simulink model "finalmodel1"  (R2024b)
(part 2 of 9)

      mask TypeOptions ModuleName: User-defined | A10Green Technology A10J-S72-175 | A10Green Technology A10J-S72-180 | A10Green Technology A10J-S72-185 | A10Green Technology A10J-M60-220 | A10Green Technology A10J-M60-225 | A10Green Technology A10J-M60-230 | A10Green Technology A10J-M60-235 | A10Green Technology A10J-M60-240 | A2Peak Power POWER ON P220-6x10 | Aavid Solar ASMS-165P | Aavid Solar ASMS-180M | Aavid Solar ASMS-185M | Aavid Solar ASMS-220P | Aavid Solar ASMS-225M | Aavid Solar ASMS-230M | Aavid Solar ASMS-235M | Aavid Solar ASMS-270P | Aavid Thermalloy ASMP-175M | Aavid Thermalloy ASMP-180M | Ablytek 5MN6C175-A0 | Ablytek 5MN6C180-A0 | Ablytek 5MN6C185-A0 | Ablytek 6PN6A220-A0 | Ablytek 6PN6A225-A0 | Ablytek 6PN6A230-A0 | Ablytek 6PN6A235-A0 | Ablytek 6PN6A240-A0 | Ablytek 6MN6A270 | Ablytek 6MN6A275 | Ablytek 6MN6A280 | Ablytek 6MN6A285 | Ablytek 6MN6A290 | AccuSolar Power ASP610-B230 | Advance Power API-P210 | Advance Power API-P215 | Advance Power API-P220 | Advance Power API-M225 | Advance Power API-P225 | Advance Power API-M230 | Advance Power API-P230 | Advance Power API-M235 | Advance Power API-P235 | Advance Power API-M240 | Advance Power API-P240 | Advance Power API-M245 | Advance Power API-P245 | Advance Power API-M250 | Advance Power API-P250 | Advance Power API-M255 | Advance Power API-P255 | Advance Power API-M260 | Advance Power API-P260 | Advance Power API-M265 | Advance Power API-P265 | Advance Power API-M270 | Advance Power API-P270 | Advance Power API-M275 | Advance Power API-P275 | Advance Power API-M280 | Advance Power API-P280 | Advance Power API-M285 | Advance Power API-P285 | Advance Power API-M290 | Advance Power API-P290 | Advance Power API-M295 | Advance Power API-P295 | Advance Power API-M300 | Advance Power API-P300 | Advance Power API-M305 | Advance Power API-P305 | Advance Power API-M310 | Advance Power API-P310 | Advance Power API-M315 | Advance Power API-P315 | Advance Power API-P320 | Advance Power API-P325 | Advance Power API-M330 | Advance Power API-P330 | Advance Power API-M335 | Advance Power API-P335 | Advance Power API-M340 | Advance Power API-M345 | Advance Power API-M350 | Advance Power API-M355 | Advance Power API-M360 | Advance Power API-M365 | Advance Power API-M370 | Advance Solar Hydro Wind Power API-150 | Advance Solar Hydro Wind Power API-160 | Advance Solar Hydro Wind Power API-165 | Advance Solar Hydro Wind Power API-170 | Advance Solar Hydro Wind Power API-175 | Advance Solar Hydro Wind Power API-180 | Advance Solar Hydro Wind Power API156P-200 | Advance Solar Hydro Wind Power API156P-210 | Advance Solar Hydro Wind Power API156P-220 | Advance Solar Hydro Wind Power API156P-230 | Advanced Renewable Energy AREi-210W-M6-G | Advanced Renewable Energy AREi-215W-M6-G | Advanced Renewable Energy AREi-220W-M6-G | Advanced Renewable Energy AREi-225W-M6-G | Advanced Renewable Energy AREi-230W-M6-G | Advanced Solar Power (Hangzhou) ASP-S1-80 | Aleo Solar P18y250 | Aleo Solar S18y250 | Aleo Solar P18y255 | Aleo Solar S18y255 | Aleo Solar P18y260 | Aleo Solar S18y260 | Aleo Solar P18Y265 | Aleo Solar S18y265 | Aleo Solar S19Y270 | Aleo Solar S79y270 | Aleo Solar P19Y275 | Aleo Solar S19y275 | Aleo Solar S79y275 | Aleo Solar S19y280 | Aleo Solar S59y280 | Aleo Solar S79y280 | Aleo Solar P19Y285 | Aleo Solar S19y285 | Aleo Solar S59y285 | Aleo Solar S79y285 | Aleo Solar P19Y290 | Aleo Solar S19y290 | Aleo Solar S59y290 | Aleo Solar S79Y290 | Aleo Solar P19Y295 | Aleo Solar S19Y295 | Aleo Solar S59Y295 | Aleo Solar S79Y295 | Aleo Solar P19Y300 | Aleo Solar S19Y300 | Aleo Solar S59Y300 | Aleo Solar S79Y300 | Aleo Solar P19Y305 | Aleo Solar S19Y305 | Aleo Solar S59Y305 | Aleo Solar S79Y305 | Aleo Solar P19Y310 | Aleo Solar S19Y310 | Aleo Solar S59Y310 | alfasolar alfasolar P6L60-220 | alfasolar alfasolar P6L60-225 | alfasolar alfasolar P6L60-230 | alfasolar alfasolar P6L60-235 | alfasolar alfasolar M6L60-240 | alfasolar alfasolar P6L60-240 | alfasolar alfasolar M6L60-245 | alfasolar alfasolar P6L60-245 | alfasolar alfasolar M6L60-250 | alfasolar alfasolar P6L60-250 | alfasolar alfasolar M6L60-255 | alfasolar alfasolar M6L60-260 | alfasolar alfasolar M6L60-265 | Alps Technology ATI-S572-175 | Alps Technology ATI-S572-180 | Alps Technology ATI-S572-185 | Alps Technology ATI-M660-220 | Alps Technology ATI-M660-225 | Alps Technology ATI-M660-230 | Alps Technology ATI-M660-235 | Alps Technology ATI-M660-240 | American Solar Wholesale ASW-175M | American Solar Wholesale ASW-180M | American Solar Wholesale ASW-185M | American Solar Wholesale ASW-215P | American Solar Wholesale ASW-220P | American Solar Wholesale ASW-225M | American Solar Wholesale ASW-225P | American Solar Wholesale ASW-230M | American Solar Wholesale ASW-230P | American Solar Wholesale ASW-235M | American Solar Wholesale ASW-235P | American Solar Wholesale ASW-240M-60 | American Solar Wholesale ASW-240P | American Solar Wholesale ASW-245M | American Solar Wholesale ASW-245P | American Solar Wholesale ASW-250M | American Solar Wholesale ASW-250P | American Solar Wholesale ASW-260M | American Solar Wholesale ASW-260P | American Solar Wholesale ASW-265M | American Solar Wholesale ASW-270M | American Solar Wholesale ASW-270P | American Solar Wholesale ASW-275M | American Solar Wholesale ASW-280M | American Solar Wholesale ASW-280P | American Solar Wholesale ASW-285M | American Solar Wholesale ASW-285P | American Solar Wholesale ASW-290M | American Solar Wholesale ASW-290P | American Solar Wholesale ASW-295M | American Solar Wholesale ASW-295P | American Solar Wholesale ASW-300M | American Solar Wholesale ASW-300P | American Solar Wholesale ASW-305P | American Solar Wholesale ASW-310P | American Solar Wholesale ASW-315P | American Value SM240-5M | American Value SM245-5M | American Value SM250-5M | American Value SM255-5M | American Value SM260-5M | Amerisolar-Worldwide Energy and Manufacturing USA Co._ Ltd AS-5M36-165W | Amerisolar-Worldwide Energy and Manufacturing USA Co._ Ltd AS-5M-170W | Amerisolar-Worldwide Energy and Manufacturing USA Co._ Ltd AS-5M36-170W | Amerisolar-Worldwide Energy and Manufacturing USA Co._ Ltd AS-6M24-170W | Amerisolar-Worldwide Energy and Manufacturing USA Co._ Ltd AS-6P24-170W | Amerisolar-Worldwide Energy and Manufacturing USA Co._ Ltd AS-5M-175W | Amerisolar-Worldwide Energy and Manufacturing USA Co._ Ltd AS-5M36-175W | Amerisolar-Worldwide Energy and Manufacturing USA Co._ Ltd AS-6M24-175W | Amerisolar-Worldwide Energy and Manufacturing USA Co._ Ltd AS-6P24-175W | Amerisolar-Worldwide Energy and Manufacturing USA Co._ Ltd AS-5M-180W | Amerisolar-Worldwide Energy and Manufacturing USA Co._ Ltd AS-5M36-180W | Amerisolar-Worldwide Energy and Manufacturing USA Co._ Ltd AS-6M24-180W | Amerisolar-Worldwide Energy and Manufacturing USA Co._ Ltd AS-6P24-180W | Amerisolar-Worldwide Energy and Manufacturing USA Co._ Ltd AS-5M-185W | Amerisolar-Worldwide Energy and Manufacturing USA Co._ Ltd AS-5M36-185W | Amerisolar-Worldwide Energy and Manufacturing USA Co._ Ltd AS-6M24-185W | Amerisolar-Worldwide Energy and Manufacturing USA Co._ Ltd AS-6P24-185W | Amerisolar-Worldwide Energy and Manufacturing USA Co._ Ltd AS-5M-190W | Amerisolar-Worldwide Energy and Manufacturing USA Co._ Ltd AS-6M24-190W | Amerisolar-Worldwide Energy and Manufacturing USA Co._ Ltd AS-6P24-190W | Amerisolar-Worldwide Energy and Manufacturing USA Co._ Ltd AS-6M27-215W | Amerisolar-Worldwide Energy and Manufacturing USA Co._ Ltd AS-6M27-B-215W | Amerisolar-Worldwide Energy and Manufacturing USA Co._ Ltd AS-6M27-220W | Amerisolar-Worldwide Energy and Manufacturing USA Co._ Ltd AS-6M27-B-220W | Amerisolar-Worldwide Energy and Manufacturing USA Co._ Ltd AS-6M30-220W | Amerisolar-Worldwide Energy and Manufacturing USA Co._ Ltd AS-6P30-220W | Amerisolar-Worldwide Energy and Manufacturing USA Co._ Ltd AS-6M27-225W | Amerisolar-Worldwide Energy and Manufacturing USA Co._ Ltd AS-6M27-B-225W | Amerisolar-Worldwide Energy and Manufacturing USA Co._ Ltd AS-6M30-225W | Amerisolar-Worldwide Energy and Manufacturing USA Co._ Ltd AS-6P30-225W | Amerisolar-Worldwide Energy and Manufacturing USA Co._ Ltd AS-6M30-230W | Amerisolar-Worldwide Energy and Manufacturing USA Co._ Ltd AS-6P30-230W | Amerisolar-Worldwide Energy and Manufacturing USA Co._ Ltd AS-6M30-235W | Amerisolar-Worldwide Energy and Manufacturing USA Co._ Ltd AS-6M30-B-235W | Amerisolar-Worldwide Energy and Manufacturing USA Co._ Ltd AS-6M27-240W | Amerisolar-Worldwide Energy and Manufacturing USA Co._ Ltd AS-6M30-240W | Amerisolar-Worldwide Energy and Manufacturing USA Co._ Ltd AS-6M30-B-240W | Amerisolar-Worldwide Energy and Manufacturing USA Co._ Ltd AS-6P30-240W | Amerisolar-Worldwide Energy and Manufacturing USA Co._ Ltd AS-6M-245W | Amerisolar-Worldwide Energy and Manufacturing USA Co._ Ltd AS-6M30-245W | Amerisolar-Worldwide Energy and Manufacturing USA Co._ Ltd AS-6M30-B-245W | Amerisolar-Worldwide Energy and Manufacturing USA Co._ Ltd AS-6P30-245W | Amerisolar-Worldwide Energy and Manufacturing USA Co._ Ltd AS-6M-250W | Amerisolar-Worldwide Energy and Manufacturing USA Co._ Ltd AS-6M30-250W | Amerisolar-Worldwide Energy and Manufacturing USA Co._ Ltd AS-6P30-250W | Amerisolar-Worldwide Energy and Manufacturing USA Co._ Ltd AS-6M30-255W | Amerisolar-Worldwide Energy and Manufacturing USA Co._ Ltd AS-6P30-255W | Amerisolar-Worldwide Energy and Manufacturing USA Co._ Ltd AS-6M30-260W | Amerisolar-Worldwide Energy and Manufacturing USA Co._ Ltd AS-6P30-260W | Amerisolar-Worldwide Energy and Manufacturing USA Co._ Ltd AS-6M-265W | Amerisolar-Worldwide Energy and Manufacturing USA Co._ Ltd AS-6M30-265W | Amerisolar-Worldwide Energy and Manufacturing USA Co._ Ltd AS-6P30-265W | Amerisolar-Worldwide Energy and Manufacturing USA Co._ Ltd AS-6M-270W | Amerisolar-Worldwide Energy and Manufacturing USA Co._ Ltd AS-6M30-270W | Amerisolar-Worldwide Energy and Manufacturing USA Co._ Ltd AS-6P30-270W | Amerisolar-Worldwide Energy and Manufacturing USA Co._ Ltd AS-6M-275W | Amerisolar-Worldwide Energy and Manufacturing USA Co._ Ltd AS-6P-275W | Amerisolar-Worldwide Energy and Manufacturing USA Co._ Ltd AS-6P30-275W | Amerisolar-Worldwide Energy and Manufacturing USA Co._ Ltd AS-6M-280W | Amerisolar-Worldwide Energy and Manufacturing USA Co._ Ltd AS-6M30-280W | Amerisolar-Worldwide Energy and Manufacturing USA Co._ Ltd AS-6M-B-280W | Amerisolar-Worldwide Energy and Manufacturing USA Co._ Ltd AS-6P-280W | Amerisolar-Worldwide Energy and Manufacturing USA Co._ Ltd AS-6P30-280W | Amerisolar-Worldwide Energy and Manufacturing USA Co._ Ltd AS-6M-285W | Amerisolar-Worldwide Energy and Manufacturing USA Co._ Ltd AS-6M30-285W | Amerisolar-Worldwide Energy and Manufacturing USA Co._ Ltd AS-6M-B-285W | Amerisolar-Worldwide Energy and Manufacturing USA Co._ Ltd AS-6P-285W | Amerisolar-Worldwide Energy and Manufacturing USA Co._ Ltd AS-6M-290W | Amerisolar-Worldwide Energy and Manufacturing USA Co._ Ltd AS-6M-B-290W | Amerisolar-Worldwide Energy and Manufacturing USA Co._ Ltd AS-6P-290W | Amerisolar-Worldwide Energy and Manufacturing USA Co._ Ltd AS-6M-295W | Amerisolar-Worldwide Energy and Manufacturing USA Co._ Ltd AS-6M-B-295W | Amerisolar-Worldwide Energy and Manufacturing USA Co._ Ltd AS-6P-295W | Amerisolar-Worldwide Energy and Manufacturing USA Co._ Ltd AS-6M-300W | Amerisolar-Worldwide Energy and Manufacturing USA Co._ Ltd AS-6P-300W | Amerisolar-Worldwide Energy and Manufacturing USA Co._ Ltd AS-6M-305W | Amerisolar-Worldwide Energy and Manufacturing USA Co._ Ltd AS-6P-305W | Amerisolar-Worldwide Energy and Manufacturing USA Co._ Ltd AS-6M-310W | Amerisolar-Worldwide Energy and Manufacturing USA Co._ Ltd AS-6P-310W | Amerisolar-Worldwide Energy and Manufacturing USA Co._ Ltd AS-6M-315W | Amerisolar-Worldwide Energy and Manufacturing USA Co._ Ltd AS-6P-315W | Amerisolar-Worldwide Energy and Manufacturing USA Co._ Ltd AS-6M-320W | Amerisolar-Worldwide Energy and Manufacturing USA Co._ Ltd AS-6P-320W | Amerisolar-Worldwide Energy and Manufacturing USA Co._ Ltd AS-6P-325W | Amerisolar-Worldwide Energy and Manufacturing USA Co._ Ltd AS-6P-330W | Amerisolar-Worldwide Energy and Manufacturing USA Co._ Ltd AS-6M-335W | Amerisolar-Worldwide Energy and Manufacturing USA Co._ Ltd AS-6P-335W | Amerisolar-Worldwide Energy and Manufacturing USA Co._ Ltd AS-6M-340W | Amerisolar-Worldwide Energy and Manufacturing USA Co._ Ltd AS-6M-345W | Amerisolar-Worldwide Energy and Manufacturing USA Co._ Ltd AS-6M-350W | Andalay Solar ST_165_1_DC0_0_B | Andalay Solar ST165-1 | Andalay Solar ST_170_1_DC0_0_B | Andalay Solar ST170-1 | Andalay Solar ST_175_1_DC0_0_B | Andalay Solar ST175-1 | Andalay Solar ST-175-1AC1-A-A | Andalay Solar ST-175-1AC3-B-A | Andalay Solar KC180-1 | Andalay Solar ST_180_1_DC0_0_B | Andalay Solar ST180-1 | Andalay Solar ST_185_1_DC0_0_B | Andalay Solar ST-185-1 | Andalay Solar ST-185-1AC1-A-A | Andalay Solar ST-185-1AC1-A-B | Andalay Solar ST-185-1AC3-B-A | Andalay Solar ST-185-1AC3-B-B | Andalay Solar ST_190_1_DC0_0_B | Andalay Solar ST-190-1AC1-A-B | Andalay Solar ST-190-1AC3-B-B | Andalay Solar ST_195_1_DC0_0_B | Andalay Solar ST-195-1AC1-A-B | Andalay Solar ST-195-1AC3-B-B | Andalay Solar KC205-1 | Andalay Solar KC210-1 | Andalay Solar LW-230-1-AC0-D-B | Andalay Solar LW-230-1-AC1-A-B | Andalay Solar LW-230-1-AC2-D-B | Andalay Solar LW-230-1-AC3-B-B | Andalay Solar LW-230-1-DC0-0-B | Andalay Solar LW-230-1-DC0-0-BL | Andalay Solar LW-230-1-DC1-0-B | Andalay Solar LW-235-1-AC0-D-B | Andalay Solar LW-235-1-AC1-A-B | Andalay Solar LW-235-1-AC2-D-B | Andalay Solar LW-235-1-AC3-B-B | Andalay Solar LW-235-1-DC0-0-B | Andalay Solar LW-235-1-DC0-0-BL | Andalay Solar LW-235-1-DC1-0-B | Andalay Solar LW-240-1-AC0-D-B | Andalay Solar LW-240-1-AC1-A-B | Andalay Solar LW-240-1-AC2-D-B | Andalay Solar LW-240-1-AC3-B-B | Andalay Solar LW-240-1-DC0-0-B | Andalay Solar LW-240-1-DC0-0-BL | Andalay Solar LW-240-1-DC1-0-B | Andalay Solar TW-240-1-AC2-D-B | Andalay Solar TW-240-1-DC4-0-B | Andalay Solar TW-245-1-AC2-D-B | Andalay Solar TW-245-1-DC4-0-B | Andalay Solar AX-250-1-DC4-0-B | Andalay Solar TW-250-1-AC2-D-B | Andalay Solar TW-250-1-DC4-0-B | Andalay Solar AX-255-1-DC4-0-B | Andalay Solar AX-260-1-DC4-0-B | Andalay Solar ST_260_1_DC0_0_B | Andalay Solar ST_270_1_DC0_0_B | Andalay Solar ST_280_1_DC0_0_B | Andalay Solar ST_290_1_DC0_0_B | Anhui Rinengzhongtian Semiconductor Development QJM160-72 | Anhui Rinengzhongtian Semiconductor Development QJM165-72 | Anhui Rinengzhongtian Semiconductor Development QJM170-72 | Anhui Rinengzhongtian Semiconductor Development QJM175-72 | Anhui Rinengzhongtian Semiconductor Development QJM180-72 | Anhui Rinengzhongtian Semiconductor Development QJM185-72 | Anhui Rinengzhongtian Semiconductor Development QJM190-72 | Anhui Rinengzhongtian Semiconductor Development QJM195-72 | Anhui Rinengzhongtian Semiconductor Development QJM200-72 | Anhui Rinengzhongtian Semiconductor Development QJP205-60 | Anhui Rinengzhongtian Semiconductor Development QJP210-60 | Anhui Rinengzhongtian Semiconductor Development QJP215-60 | Anhui Rinengzhongtian Semiconductor Development QJM220-60 | Anhui Rinengzhongtian Semiconductor Development QJP220-60 | Anhui Rinengzhongtian Semiconductor Development QJM225-60 | Anhui Rinengzhongtian Semiconductor Development QJP225-60 | Anhui Rinengzhongtian Semiconductor Development QJM230-60 | Anhui Rinengzhongtian Semiconductor Development QJP230-60 | Anhui Rinengzhongtian Semiconductor Development QJM235-60 | Anhui Rinengzhongtian Semiconductor Development QJP235-60 | Anhui Rinengzhongtian Semiconductor Development QJM240-60 | Anhui Rinengzhongtian Semiconductor Development QJP240-60 | Anhui Rinengzhongtian Semiconductor Development QJM245-60 | Anhui Rinengzhongtian Semiconductor Development QJP245-60 | Anhui Rinengzhongtian Semiconductor Development QJM250-60 | Anhui Rinengzhongtian Semiconductor Development QJP250-60 | Anhui Rinengzhongtian Semiconductor Development QJM255-60 | Anhui Rinengzhongtian Semiconductor Development QJP255-60 | Anhui Rinengzhongtian Semiconductor Development QJP255-72 | Anhui Rinengzhongtian Semiconductor Development QJM260-60 | Anhui Rinengzhongtian Semiconductor Development QJP260-60 | Anhui Rinengzhongtian Semiconductor Development QJP260-72 | Anhui Rinengzhongtian Semiconductor Development QJM265-60 | Anhui Rinengzhongtian Semiconductor Development QJP265-60 | Anhui Rinengzhongtian Semiconductor Development QJP265-72 | Anhui Rinengzhongtian Semiconductor Development QJM270-60 | Anhui Rinengzhongtian Semiconductor Development QJM270-72 | Anhui Rinengzhongtian Semiconductor Development QJP270-60 | Anhui Rinengzhongtian Semiconductor Development QJP270-72 | Anhui Rinengzhongtian Semiconductor Development QJM275-60 | Anhui Rinengzhongtian Semiconductor Development QJM275-72 | Anhui Rinengzhongtian Semiconductor Development QJP275-60 | Anhui Rinengzhongtian Semiconductor Development QJP275-72 | Anhui Rinengzhongtian Semiconductor Development QJM280-72 | Anhui Rinengzhongtian Semiconductor Development QJP280-72 | Anhui Rinengzhongtian Semiconductor Development QJM285-72 | Anhui Rinengzhongtian Semiconductor Development QJP285-72 | Anhui Rinengzhongtian Semiconductor Development QJM290-72 | Anhui Rinengzhongtian Semiconductor Development QJP290-72 | Anhui Rinengzhongtian Semiconductor Development QJM295-72 | Anhui Rinengzhongtian Semiconductor Development QJP295-72 | Anhui Rinengzhongtian Semiconductor Development QJP300-72 | Anhui Rinengzhongtian Semiconductor Development QJM305-72 | Anhui Rinengzhongtian Semiconductor Development QJP305-72 | Anhui Rinengzhongtian Semiconductor Development QJM310-72 | Anhui Rinengzhongtian Semiconductor Development QJP310-72 | Anhui Rinengzhongtian Semiconductor Development QJM315-72 | Anhui Rinengzhongtian Semiconductor Development QJP315-72 | Anhui Rinengzhongtian Semiconductor Development QJM320-72 | Anhui Rinengzhongtian Semiconductor Development QJP320-72 | Anhui Rinengzhongtian Semiconductor Development QJM325-72 | Anhui Rinengzhongtian Semiconductor Development QJP325-72 | Anhui Rinengzhongtian Semiconductor Development QJM330-72 | Anhui Rinengzhongtian Semiconductor Development QJP330-72 | Anhui Rinengzhongtian Semiconductor Development Co._ Ltd QJM335-72 | Anhui Rinengzhongtian Semiconductor Development Co._ Ltd QJM340-72 | Anhui Rinengzhongtian Semiconductor Development Co._ Ltd QJM345-72 | Anhui Rinengzhongtian Semiconductor Development Co._ Ltd QJM350-72 | Anhui Rinengzhongtian Semiconductor Development Co._ Ltd QJM355-72 | Anhui Rinengzhongtian Semiconductor Development Co._ Ltd QJM360-72 | Anhui Rinengzhongtian Semiconductor Development Co._ Ltd QJM365-72 | Anhui Rinengzhongtian Semiconductor Development Co._ Ltd QJM370-72 | Anji Dasol Solar Energy Science & Technology DS-A4-210 | Anji Dasol Solar Energy Science & Technology DS-A4-215 | Anji Dasol Solar Energy Science & Technology DS-A4-220 | Anji Dasol Solar Energy Science & Technology DS-A4-225 | Anji Dasol Solar Energy Science & Technology DS-A4-230 | Anji Technology AJP-S572-175 | Anji Technology AJP-S572-180 | Anji Technology AJP-S572-185 | Anji Technology AJP-M660-220 | Anji Technology AJP-M660-225 | Anji Technology AJP-M660-230 | Anji Technology AJP-M660-235 | Anji Technology AJP-M660-240 | Anji Technology AJP-M660-245 | Anji Technology AJP-M660-250 | Antaris Solar AS P 230 | Antaris Solar SM-230PC8 | Antaris Solar SM-235PC8 | Antaris Solar SM-240PC8 | Antaris Solar SM-245PC8 | Antaris Solar SM-250PC8 | Antaris Solar SM-275PC8 | Antaris Solar SM-280PC8 | Antaris Solar SM-285PC8 | Antaris Solar SM-290PC8 | Antaris Solar SM-295PC8 | Aplus Energy AP-PVROOF-314 | Aplus Energy AP-PVROOF-310 | Aplus Energy AP-PVROOF-319 | Aplus Energy AP-PVROOF-524 | Aplus Energy AP-PVROOF-523 | Aplus Energy AP-PVROOF-522 | Apollo Solar Energy ASEC-120G6M | Apollo Solar Energy ASEC-125G6M | Apollo Solar Energy ASEC-125G6S | Apollo Solar Energy ASEC-130G6M | Apollo Solar Energy ASEC-130G6S | Apollo Solar Energy ASEC-135G6M | Apollo Solar Energy ASEC-135G6S | Apollo Solar Energy ASEC-140G6M | Apollo Solar Energy ASEC-140G6S | Apollo Solar Energy ASEC-145G6M49 | Apollo Solar Energy ASEC-145G6S49 | Apollo Solar Energy ASEC-150G6M49 | Apollo Solar Energy ASEC-150G6S49 | Apollo Solar Energy ASEC-155G6M49 | Apollo Solar Energy ASEC-155G6S49 | Apollo Solar Energy ASEC-175G6M | Apollo Solar Energy ASEC-175G6S | Apollo Solar Energy ASEC-180G6M | Apollo Solar Energy ASEC-180G6S | Apollo Solar Energy ASEC-185G6M | Apollo Solar Energy ASEC-185G6S | Apollo Solar Energy ASEC-190G6M | Apollo Solar Energy ASEC-190G6M68 | Apollo Solar Energy ASEC-190G6S | Apollo Solar Energy ASEC-190G6S68 | Apollo Solar Energy ASEC-195G6M | Apollo Solar Energy ASEC-195G6M68 | Apollo Solar Energy ASEC-195G6S | Apollo Solar Energy ASEC-195G6S68 | Apollo Solar Energy ASEC-200G6M | Apollo Solar Energy ASEC-200G6M68 | Apollo Solar Energy ASEC-200G6S | Apollo Solar Energy ASEC-200G6S68 | Apollo Solar Energy ASEC-205G6M | Apollo Solar Energy ASEC-205G6M68 | Apollo Solar Energy ASEC-205G6S | Apollo Solar Energy ASEC-205G6S68 | Apollo Solar Energy ASEC-210G6M | Apollo Solar Energy ASEC-210G6M68 | Apollo Solar Energy ASEC-210G6S | Apollo Solar Energy ASEC-210G6S68 | Apollo Solar Energy ASEC-215G6M | Apollo Solar Energy ASEC-215G6M68 | Apollo Solar Energy ASEC-215G6M69 | Apollo Solar Energy ASEC-215G6S | Apollo Solar Energy ASEC-215G6S68 | Apollo Solar Energy ASEC-215G6S69 | Apollo Solar Energy ASEC-220G6M | Apollo Solar Energy ASEC-220G6M68 | Apollo Solar Energy ASEC-220G6M69 | Apollo Solar Energy ASEC-220G6S | Apollo Solar Energy ASEC-220G6S68 | Apollo Solar Energy ASEC-220G6S69 | Apollo Solar Energy ASEC-225G6M | Apollo Solar Energy ASEC-225G6M69 | Apollo Solar Energy ASEC-225G6S | Apollo Solar Energy ASEC-225G6S69 | Apollo Solar Energy ASEC-230G6M | Apollo Solar Energy ASEC-230G6M69 | Apollo Solar Energy ASEC-230G6S | Apollo Solar Energy ASEC-230G6S69 | Apollo Solar Energy ASEC-235G6M | Apollo Solar Energy ASEC-235G6M69 | Apollo Solar Energy ASEC-235G6S | Apollo Solar Energy ASEC-235G6S69 | Apollo Solar Energy ASEC-240G6M69 | Apollo Solar Energy ASEC-240G6M6A | Apollo Solar Energy ASEC-240G6S69 | Apollo Solar Energy ASEC-240G6S6A | Apollo Solar Energy ASEC-245G6M | Apollo Solar Energy ASEC-245G6M69 | Apollo Solar Energy ASEC-245G6M6A | Apollo Solar Energy ASEC-245G6S69 | Apollo Solar Energy ASEC-245G6S6A | Apollo Solar Energy ASEC-250G6M | Apollo Solar Energy ASEC-250G6M6A | Apollo Solar Energy ASEC-250G6M6B | Apollo Solar Energy ASEC-250G6S6A | Apollo Solar Energy ASEC-250G6S6B | Apollo Solar Energy ASEC-255G6M | Apollo Solar Energy ASEC-255G6M6A | Apollo Solar Energy ASEC-255G6M6B | Apollo Solar Energy ASEC-255G6S | Apollo Solar Energy ASEC-255G6S6A | Apollo Solar Energy ASEC-255G6S6B | Apollo Solar Energy ASEC-260G6M | Apollo Solar Energy ASEC-260G6M6A | Apollo Solar Energy ASEC-260G6M6B | Apollo Solar Energy ASEC-260G6S | Apollo Solar Energy ASEC-260G6S6A | Apollo Solar Energy ASEC-260G6S6B | Apollo Solar Energy ASEC-265G6M | Apollo Solar Energy ASEC-265G6M6A | Apollo Solar Energy ASEC-265G6M6B | Apollo Solar Energy ASEC-265G6S | Apollo Solar Energy ASEC-265G6S6A | Apollo Solar Energy ASEC-265G6S6B | Apollo Solar Energy ASEC-270G6M | Apollo Solar Energy ASEC-270G6M6A | Apollo Solar Energy ASEC-270G6M6B | Apollo Solar Energy ASEC-270G6S | Apollo Solar Energy ASEC-270G6S6A | Apollo Solar Energy ASEC-270G6S6B | Apollo Solar Energy ASEC-275G6M | Apollo Solar Energy ASEC-275G6M6B | Apollo Solar Energy ASEC-275G6S | Apollo Solar Energy ASEC-275G6S6B | Apollo Solar Energy ASEC-280G6M | Apollo Solar Energy ASEC-280G6M6B | Apollo Solar Energy ASEC-280G6S | Apollo Solar Energy ASEC-280G6S6B | Apollo Solar Energy ASEC-285G6M | Apollo Solar Energy ASEC-285G6M6B | Apollo Solar Energy ASEC-285G6S | Apollo Solar Energy ASEC-285G6S6B | Apollo Solar Energy ASEC-290G6M | Apollo Solar Energy ASEC-290G6M6B | Apollo Solar Energy ASEC-290G6S | Apollo Solar Energy ASEC-290G6S6B | Apollo Solar Energy ASEC-295G6M | Apollo Solar Energy ASEC-295G6M6B | Apollo Solar Energy ASEC-295G6S | Apollo Solar Energy ASEC-295G6S6B | Apollo Solar Energy ASEC-300G6M | Apollo Solar Energy ASEC-300G6S | Apollo Solar Energy ASEC-305G6M | Apollo Solar Energy ASEC-305G6S | Apollo Solar Energy ASEC-310G6M | Apollo Solar Energy ASEC-310G6S | Apollo Solar Energy ASEC-315G6M | Apollo Solar Energy ASEC-315G6S | Apollo Solar Energy ASEC-320G6M | Apollo Solar Energy ASEC-320G6S | Apollo Solar Energy ASEC-325G6M | Apollo Solar Energy ASEC-325G6S | APOS Energy AP130 | APOS Energy AP135 | APOS Energy AS135 | APOS Energy AP140 | APOS Energy AS140 | APOS Energy AS145 | APOS Energy AP175 | APOS Energy AP180 | APOS Energy AS180 | APOS Energy AP185 | APOS Energy AS185 | APOS Energy AP190 | APOS Energy AS190 | APOS Energy AP195 | APOS Energy AS195 | APOS Energy AP 200M | APOS Energy AP200 | APOS Energy AS200 | APOS Energy AP 205M | APOS Energy AP205 | APOS Energy AS205 | APOS Energy AP 210M | APOS Energy AP210 | APOS Energy AS210 | APOS Energy AP 215M | APOS Energy AP215 | APOS Energy AS215 | APOS Energy AP 220M | APOS Energy AP220 | APOS Energy AS220 | APOS Energy AP 225M | APOS Energy AP225 | APOS Energy AS225 | APOS Energy AP 230M | APOS Energy AP230 | APOS Energy AS230 | APOS Energy AP 235M | APOS Energy AS235 | APOS Energy AP 240M | APOS Energy AS240 | Applied Materials 1/4 Size Tandem Junction | Applied Materials 1/4 Size Single Junction Version 1.0 | Applied Materials 1/2-L Size Single Junction Version 1.0 | Applied Materials 1/2-P Size Single Junction Version 1.0 | Applied Materials 1/2-L Size Tandem Junction | Applied Materials 1/2-P Size Tandem Junction | Applied Materials Full Size Single Junction Version 1.0 | Applied Materials Full Size Tandem Junction | Applied Quantum Technology AQT125MA-160W | Applied Quantum Technology AQT125MA-165W | Applied Quantum Technology AQT125MA-170W | Applied Quantum Technology AQT125MA-175W | Applied Quantum Technology AQT125MA-180W | Applied Quantum Technology AQT156PA-190W | Applied Quantum Technology AQT156PA-195W | Applied Quantum Technology AQT156PA-200W | Applied Quantum Technology AQT156PA-205W | Applied Quantum Technology AQT156PA-210W | Applied Quantum Technology AQT156PA-215W | Applied Quantum Technology AQT156PA-220W | Applied Quantum Technology AQT156PA-225W | Applied Quantum Technology AQT156PA-230W | Armageddon Energy SolarClover Dual Module | Astronergy Solarmodule ASM6610P 250 | Astronergy Solarmodule ASM6610P 255 | Astronergy Solarmodule ASM6610P 260 | Astronergy Solarmodule ASM6610P 265 | Astronergy Solarmodule ASM6610P 270 | Astronergy Solarmodule ASM6612P 295 | Astronergy Solarmodule ASM6612P 300 | Astronergy Solarmodule ASM6612P 305 | Astronergy Solarmodule ASM6612P 310 | Astronergy Solarmodule ASM6612P 315 | Astronergy Solarmodule ASM6612P 320 | ASUN Energy ASM190PCA0G101 | ASUN Energy ASM195PCA0G101 | ASUN Energy ASM200PCA0G101 | ASUN Energy ASM205PCA0G101 | ASUN Energy ASM210PCA0G101 | Atersa (Aplicaciones Tecnicas de la Energia) A-225P | Atersa (Aplicaciones Tecnicas de la Energia) A-230P | Atersa (Aplicaciones Tecnicas de la Energia) A-235P | Atersa (Aplicaciones Tecnicas de la Energia) A-240P | Atersa (Aplicaciones Tecnicas de la Energia) A-245P | Atersa (Aplicaciones Tecnicas de la Energia) A-250P | Atersa (Aplicaciones Tecnicas de la Energia) A-275P | Atersa (Aplicaciones Tecnicas de la Energia) A-280P | Atersa (Aplicaciones Tecnicas de la Energia) A-285P | Atersa (Aplicaciones Tecnicas de la Energia) A-290P | Atersa (Aplicaciones Tecnicas de la Energia) A-295P | Atersa (Aplicaciones Tecnicas de la Energia) A-300P | Atlantis Energy AES-SS-100-C | Atlantis Energy AES-SS-100-W | Atlantis Energy Systems SS125LM | Atlantis Energy Systems SS125GM | Atlantis Energy Systems SS156LM | Atlantis Energy Systems SS156GM | Atlantis Energy Systems TS125LM | Atlantis Energy Systems TS125GM | Atlantis Energy Systems TS125SM | Atlantis Energy Systems TS125SM-IEC | Atlantis Energy Systems TSG156LM | Atlantis Energy Systems TSG156GM | AU Optronics PM180M00.0_170 | AU Optronics PM180M00.0_175 | AU Optronics PM180M00.0_180 | AU Optronics PM200M00_190 | AU Optronics PM200M00_195 | AU Optronics PM200M00_200 | AU Optronics PM200M00_205 | AU Optronics PM200M00_210 | AU Optronics PM220P00_215 | AU Optronics PM220P02.0_215 | AU Optronics PM220P00.4_220 | AU Optronics PM220P00_220 | AU Optronics PM220P01.0_220 | AU Optronics PM220P02.0_220 | AU Optronics PM060P00_225 | AU Optronics PM060P01_225 | AU Optronics PM060P02_225 | AU Optronics PM060PB0_225 | AU Optronics PM060PB1_225 | AU Optronics PM060PBR_225 | AU Optronics PM060PW0_225 | AU Optronics PM060PW1_225 | AU Optronics PM060PW8_225 | AU Optronics PM060PWR_225 | AU Optronics PM220P00.4_225 | AU Optronics PM220P00_225 | AU Optronics PM220P01.0_225 | AU Optronics PM220P02.0_225 | AU Optronics PM245P00_225 | AU Optronics PM060P00_230 | AU Optronics PM060P01_230 | AU Optronics PM060P02_230 | AU Optronics PM060PB0_230 | AU Optronics PM060PB1_230 | AU Optronics PM060PBR_230 | AU Optronics PM060PW0_230 | AU Optronics PM060PW1_230 | AU Optronics PM060PW8_230 | AU Optronics PM060PWR_230 | AU Optronics PM220P00.4_230 | AU Optronics PM220P00_230 | AU Optronics PM220P01.0_230 | AU Optronics PM220P02.0_230 | AU Optronics PM240P00_230 | AU Optronics PM245P00_230 | AU Optronics PM245P01_230 | AU Optronics PM060P00_235 | AU Optronics PM060P01_235 | AU Optronics PM060P02_235 | AU Optronics PM060PA0_235 | AU Optronics PM060PA1_235 | AU Optronics PM060PA2_235 | AU Optronics PM060PB0_235 | AU Optronics PM060PB1_235 | AU Optronics PM060PBR_235 | AU Optronics PM060PW0_235 | AU Optronics PM060PW1_235 | AU Optronics PM060PW8_235 | AU Optronics PM060PWR_235 | AU Optronics PM220P00.4_235 | AU Optronics PM220P00_235 | AU Optronics PM220P01.0_235 | AU Optronics PM240P00_235 | AU Optronics PM240PA0_235 | AU Optronics PM245P00_235 | AU Optronics PM245P01_235 | AU Optronics PM245PA0_235 | AU Optronics PM245PA1_235 | AU Optronics PM245PA2_235 | AU Optronics PM060MA0_240 | AU Optronics PM060MA1_240 | AU Optronics PM060MA2_240 | AU Optronics PM060MBR_240 | AU Optronics PM060MWR_240 | AU Optronics PM060P00_240 | AU Optronics PM060P01_240 | AU Optronics PM060P02_240 | AU Optronics PM060PA0_240 | AU Optronics PM060PA1_240 | AU Optronics PM060PA2_240 | AU Optronics PM060PB0_240 | AU Optronics PM060PB1_240 | AU Optronics PM060PBR_240 | AU Optronics PM060PW0_240 | AU Optronics PM060PW1_240 | AU Optronics PM060PW8_240 | AU Optronics PM060PWR_240 | AU Optronics PM220P01.0_240 | AU Optronics PM240P00_240 | AU Optronics PM240PA0_240 | AU Optronics PM245P00_240 | AU Optronics PM245P01_240 | AU Optronics PM245PA0_240 | AU Optronics PM245PA1_240 | AU Optronics PM245PA2_240 | AU Optronics PM250M00_240 | AU Optronics PM250M02_240 | AU Optronics PM250MA0_240 | AU Optronics PM250MA1_240 | AU Optronics PM250MA2_240 | AU Optronics PM060MA0_245 | AU Optronics PM060MA1_245 | AU Optronics PM060MA2_245 | AU Optronics PM060MBR_245 | AU Optronics PM060MWR_245 | AU Optronics PM060P00_245 | AU Optronics PM060P01_245 | AU Optronics PM060P02_245 | AU Optronics PM060PA0_245 | AU Optronics PM060PA1_245 | AU Optronics PM060PA2_245 | AU Optronics PM060PB0_245 | AU Optronics PM060PB1_245 | AU Optronics PM060PBR_245 | AU Optronics PM060PW0_245 | AU Optronics PM060PW1_245 | AU Optronics PM060PW8_245 | AU Optronics PM060PWR_245 | AU Optronics PM240P00_245 | AU Optronics PM240PA0_245 | AU Optronics PM245P00_245 | AU Optronics PM245P01_245 | AU Optronics PM245PA0_245 | AU Optronics PM245PA1_245 | AU Optronics PM245PA2_245 | AU Optronics PM250M00_245 | AU Optronics PM250MA0_245 | AU Optronics PM250MA1_245 | AU Optronics PM250MA2_245 | AU Optronics PM060M00_250 | AU Optronics PM060M01_250 | AU Optronics PM060M02_250 | AU Optronics PM060MA0_250 | AU Optronics PM060MA1_250 | AU Optronics PM060MA2_250 | AU Optronics PM060MB0_250 | AU Optronics PM060MB1_250 | AU Optronics PM060MB2_250 | AU Optronics PM060MB3_250 | AU Optronics PM060MBR_250 | AU Optronics PM060MW0_250 | AU Optronics PM060MW1_250 | AU Optronics PM060MW2_250 | AU Optronics PM060MW3_250 | AU Optronics PM060MWR_250 | AU Optronics PM060P00_250 | AU Optronics PM060P01_250 | AU Optronics PM060P02_250 | AU Optronics PM060PA0_250 | AU Optronics PM060PA1_250 | AU Optronics PM060PA2_250 | AU Optronics PM060PB0_250 | AU Optronics PM060PB1_250 | AU Optronics PM060PBR_250 | AU Optronics PM060PW0_250 | AU Optronics PM060PW1_250 | AU Optronics PM060PW8_250 | AU Optronics PM060PWR_250 | AU Optronics PM245P00_250 | AU Optronics PM245P01_250 | AU Optronics PM245PA0_250 | AU Optronics PM245PA1_250 | AU Optronics PM245PA2_250 | AU Optronics PM250M00_250 | AU Optronics PM250M01_250 | AU Optronics PM250MA0_250 | AU Optronics PM250MA1_250 | AU Optronics PM250MA2_250 | AU Optronics PM060M00_255 | AU Optronics PM060M01_255 | AU Optronics PM060M02_255 | AU Optronics PM060MA0_255 | AU Optronics PM060MA1_255 | AU Optronics PM060MA2_255 | AU Optronics PM060MB0_255 | AU Optronics PM060MB1_255 | AU Optronics PM060MB2_255 | AU Optronics PM060MB3_255 | AU Optronics PM060MBR_255 | AU Optronics PM060MW0_255 | AU Optronics PM060MW1_255 | AU Optronics PM060MW2_255 | AU Optronics PM060MW3_255 | AU Optronics PM060MWR_255 | AU Optronics PM060P00_255 | AU Optronics PM060P01_255 | AU Optronics PM060P02_255 | AU Optronics PM060PA0_255 | AU Optronics PM060PA1_255 | AU Optronics PM060PA2_255 | AU Optronics PM060PB0_255 | AU Optronics PM060PB1_255 | AU Optronics PM060PBR_255 | AU Optronics PM060PW0_255 | AU Optronics PM060PW1_255 | AU Optronics PM060PW8_255 | AU Optronics PM060PWR_255 | AU Optronics PM245P00_255 | AU Optronics PM245P01_255 | AU Optronics PM245PA0_255 | AU Optronics PM245PA1_255 | AU Optronics PM245PA2_255 | AU Optronics PM250M00_255 | AU Optronics PM250M01_255 | AU Optronics PM250MA0_255 | AU Optronics PM250MA1_255 | AU Optronics PM250MA2_255 | AU Optronics PM060M00_260 | AU Optronics PM060M01_260 | AU Optronics PM060M02_260 | AU Optronics PM060MA0_260 | AU Optronics PM060MA1_260 | AU Optronics PM060MA2_260 | AU Optronics PM060MB0_260 | AU Optronics PM060MB1_260 | AU Optronics PM060MB2_260 | AU Optronics PM060MB3_260 | AU Optronics PM060MBR_260 | AU Optronics PM060MW0_260 | AU Optronics PM060MW1_260 | AU Optronics PM060MW2_260 | AU Optronics PM060MW3_260 | AU Optronics PM060MWR_260 | AU Optronics PM060P00_260 | AU Optronics PM060P01_260 | AU Optronics PM060P02_260 | AU Optronics PM060PA0_260 | AU Optronics PM060PA1_260 | AU Optronics PM060PA2_260 | AU Optronics PM060PB0_260 | AU Optronics PM060PB1_260 | AU Optronics PM060PBR_260 | AU Optronics PM060PW0_260 | AU Optronics PM060PW1_260 | AU Optronics PM060PW8_260 | AU Optronics PM060PWR_260 | AU Optronics PM245P00_260 | AU Optronics PM245P01_260 | AU Optronics PM245PA0_260 | AU Optronics PM245PA1_260 | AU Optronics PM245PA2_260 | AU Optronics PM250M00_260 | AU Optronics PM250M01_260 | AU Optronics PM250MA0_260 | AU Optronics PM250MA1_260 | AU Optronics PM250MA2_260 | AU Optronics PM060M00_265 | AU Optronics PM060M01_265 | AU Optronics PM060M02_265 | AU Optronics PM060MA0_265 | AU Optronics PM060MA1_265 | AU Optronics PM060MA2_265 | AU Optronics PM060MB0_265 | AU Optronics PM060MB1_265 | AU Optronics PM060MB2_265 | AU Optronics PM060MB3_265 | AU Optronics PM060MBR_265 | AU Optronics PM060MW0_265 | AU Optronics PM060MW1_265 | AU Optronics PM060MW2_265 | AU Optronics PM060MW3_265 | AU Optronics PM060MWR_265 | AU Optronics PM060PWR_265 | AU Optronics PM250M00_265 | AU Optronics PM250M01_265 | AU Optronics PM250MA0_265 | AU Optronics PM250MA1_265 | AU Optronics PM250MA2_265 | AU Optronics PM060M00_270 | AU Optronics PM060M01_270 | AU Optronics PM060M02_270 | AU Optronics PM060MA0_270 | AU Optronics PM060MA1_270 | AU Optronics PM060MA2_270 | AU Optronics PM060MB0_270 | AU Optronics PM060MB1_270 | AU Optronics PM060MB2_270 | AU Optronics PM060MB3_270 | AU Optronics PM060MBR_270 | AU Optronics PM060MW0_270 | AU Optronics PM060MW1_270 | AU Optronics PM060MW2_270 | AU Optronics PM060MW3_270 | AU Optronics PM060MWR_270 | AU Optronics PM060PWR_270 | AU Optronics PM072PB0_270 | AU Optronics PM072PB1_270 | AU Optronics PM072PBR_270 | AU Optronics PM072PW0_270 | AU Optronics PM072PW1_270 | AU Optronics PM072PWR_270 | AU Optronics PM250M00_270 | AU Optronics PM250M01_270 | AU Optronics PM250MA0_270 | AU Optronics PM250MA1_270 | AU Optronics PM250MA2_270 | AU Optronics PM300P00_270 | AU Optronics PM060M00_275 | AU Optronics PM060M01_275 | AU Optronics PM060M02_275 | AU Optronics PM060MA0_275 | AU Optronics PM060MA1_275 | AU Optronics PM060MA2_275 | AU Optronics PM060MB0_275 | AU Optronics PM060MB1_275 | AU Optronics PM060MB2_275 | AU Optronics PM060MB3_275 | AU Optronics PM060MBR_275 | AU Optronics PM060MW0_275 | AU Optronics PM060MW1_275 | AU Optronics PM060MW2_275 | AU Optronics PM060MW3_275 | AU Optronics PM060MWR_275 | AU Optronics PM060PWR_275 | AU Optronics PM072PB0_275 | AU Optronics PM072PB1_275 | AU Optronics PM072PBR_275 | AU Optronics PM072PW0_275 | AU Optronics PM072PW1_275 | AU Optronics PM072PWR_275 | AU Optronics PM250M01_275 | AU Optronics PM250MA0_275 | AU Optronics PM250MA1_275 | AU Optronics PM250MA2_275 | AU Optronics PM300P00_275 | AU Optronics PM060M00_280 | AU Optronics PM060M01_280 | AU Optronics PM060M02_280 | AU Optronics PM060MB0_280 | AU Optronics PM060MB1_280 | AU Optronics PM060MB2_280 | AU Optronics PM060MB3_280 | AU Optronics PM060MBR_280 | AU Optronics PM060MW0_280 | AU Optronics PM060MW1_280 | AU Optronics PM060MW2_280 | AU Optronics PM060MW3_280 | AU Optronics PM060MWR_280 | AU Optronics PM060PWR_280 | AU Optronics PM072PB0_280 | AU Optronics PM072PB1_280 | AU Optronics PM072PBR_280 | AU Optronics PM072PW0_280 | AU Optronics PM072PW1_280 | AU Optronics PM072PWR_280 | AU Optronics PM250M01_280 | AU Optronics PM300P00_280 | AU Optronics PM060M00_285 | AU Optronics PM060M01_285 | AU Optronics PM060M02_285 | AU Optronics PM060MB0_285 | AU Optronics PM060MB1_285 | AU Optronics PM060MB2_285 | AU Optronics PM060MB3_285 | AU Optronics PM060MBR_285 | AU Optronics PM060MW0_285 | AU Optronics PM060MW1_285 | AU Optronics PM060MW2_285 | AU Optronics PM060MW3_285 | AU Optronics PM060MWR_285 | AU Optronics PM072PB0_285 | AU Optronics PM072PB1_285 | AU Optronics PM072PBR_285 | AU Optronics PM072PW0_285 | AU Optronics PM072PW1_285 | AU Optronics PM072PWR_285 | AU Optronics PM250M01_285 | AU Optronics PM300P00_285 | AU Optronics PM060M00_290 | AU Optronics PM060M01_290 | AU Optronics PM060M02_290 | AU Optronics PM060MB0_290 | AU Optronics PM060MB1_290 | AU Optronics PM060MB2_290 | AU Optronics PM060MB3_290 | AU Optronics PM060MBR_290W | AU Optronics PM060MW0_290 | AU Optronics PM060MW1_290 | AU Optronics PM060MW2_290 | AU Optronics PM060MW3_290 | AU Optronics PM060MWR_290W | AU Optronics PM072MB0_290 | AU Optronics PM072MW0_290 | AU Optronics PM072PB0_290 | AU Optronics PM072PB1_290 | AU Optronics PM072PBR_290 | AU Optronics PM072PW0_290 | AU Optronics PM072PW1_290 | AU Optronics PM072PWR_290 | AU Optronics PM250M01_290 | AU Optronics PM300P00_290 | AU Optronics PM060MBR_295W | AU Optronics PM060MW0_295 | AU Optronics PM060MWR_295W | AU Optronics PM072MB0_295 | AU Optronics PM072MW0_295 | AU Optronics PM072PB0_295 | AU Optronics PM072PB1_295 | AU Optronics PM072PBR_295 | AU Optronics PM072PW0_295 | AU Optronics PM072PW1_295 | AU Optronics PM072PWR_295 | AU Optronics PM300P00_295 | AU Optronics PM060MBR_300W | AU Optronics PM060MW0_300 | AU Optronics PM060MWR_300W | AU Optronics PM072MB0_300 | AU Optronics PM072MW0_300 | AU Optronics PM072PB0_300 | AU Optronics PM072PB1_300 | AU Optronics PM072PBR_300 | AU Optronics PM072PW0_300 | AU Optronics PM072PW1_300 | AU Optronics PM072PWR_300 | AU Optronics PM300P00_300 | AU Optronics PM096B00_303 | AU Optronics PM060MBR_305W | AU Optronics PM060MW0_305 | AU Optronics PM060MWR_305W | AU Optronics PM072MB0_305 | AU Optronics PM072MW0_305 | AU Optronics PM072PB0_305 | AU Optronics PM072PB1_305 | AU Optronics PM072PBR_305 | AU Optronics PM072PW0_305 | AU Optronics PM072PW1_305 | AU Optronics PM072PWR_305 | AU Optronics PM096B00_305 | AU Optronics PM300P00_305 | AU Optronics PM096B00_308 | AU Optronics PM060MW0_310 | AU Optronics PM072MB0_310 | AU Optronics PM072MW0_310 | AU Optronics PM072PB0_310 | AU Optronics PM072PB1_310 | AU Optronics PM072PBR_310 | AU Optronics PM072PW0_310 | AU Optronics PM072PW1_310 | AU Optronics PM072PWR_310 | AU Optronics PM096B00_310 | AU Optronics PM300P00_310 | AU Optronics PM096B00_313 | AU Optronics PM060MW0_315 | AU Optronics PM072MB0_315 | AU Optronics PM072MW0_315 | AU Optronics PM072PB0_315 | AU Optronics PM072PB1_315 | AU Optronics PM072PBR_315 | AU Optronics PM072PW0_315 | AU Optronics PM072PW1_315 | AU Optronics PM072PWR_315 | AU Optronics PM096B00_315 | AU Optronics PM300P00_315 | AU Optronics PM096B00_318 | AU Optronics PM072MB0_320 | AU Optronics PM072MW0_320 | AU Optronics PM072PW0_320 | AU Optronics PM096B00_320 | AU Optronics PM096B00_323 | AU Optronics PM072MB0_325 | AU Optronics PM072MW0_325 | AU Optronics PM072PW0_325 | AU Optronics PM096B00_325 | AU Optronics PM096B00_327 | AU Optronics PM072MB0_330 | AU Optronics PM072MW0_330 | AU Optronics PM072PW0_330 | AU Optronics PM096B00_330 | AU Optronics PM096B00_333 | AU Optronics PM072MB0_335 | AU Optronics PM072MW0_335 | AU Optronics PM072PW0_335 | AU Optronics PM072MB0_340 | AU Optronics PM072MW0_340 | AU Optronics PM072MW0_345W | AU Optronics PM072MW0_350W | AU Optronics PM072MW0_355W | AU Optronics PM072MW0_360W | AU Optronics PM072MW0_365W | Auria Solar M115000 | Auria Solar M120000 | Auria Solar M125000 | Auxin Solar AXN6M409T130 | Auxin Solar AXN6M409T135 | Auxin Solar AXN6M409T140 | Auxin Solar AXN6M409T145 | Auxin Solar AXN6M409T150 | Auxin Solar AXN6M409T155 | Auxin Solar AXN-P6T160 | Auxin Solar AXN-M5T165 | Auxin Solar AXN-P6T165 | Auxin Solar AXN-M5T170 | Auxin Solar AXN-P6T170 | Auxin Solar AXN-M5T175 | Auxin Solar AXN-P6T175 | Auxin Solar AXN-M5T180 | Auxin Solar AXN-P6T180 | Auxin Solar AXN-P6T190 | Auxin Solar AXN-P6T195 | Auxin Solar AXN-P6T200 | Auxin Solar AXN-P6T205 | Auxin Solar AXN6P610T210 | Auxin Solar AXN-P6T210 | Auxin Solar AXN6P610T215 | Auxin Solar AXN-P6T215 | Auxin Solar AXN6P610T220 | Auxin Solar AXN-P6T220 | Auxin Solar AXN6M610T225 | Auxin Solar AXN6P610T225 | Auxin Solar AXN-P6T225 | Auxin Solar AXN6M610T230 | Auxin Solar AXN6P610T230 | Auxin Solar AXN-P6T230 | Auxin Solar AXN6M610T235 | Auxin Solar AXN6P610T235 | Auxin Solar AXN-P6T235 | Auxin Solar AXN6M610T240 | Auxin Solar AXN6P610T240 | Auxin Solar AXN-P6T240 | Auxin Solar AXN6M610T245 | Auxin Solar AXN6P610T245 | Auxin Solar AXN-P6T245 | Auxin Solar AXN6M610T250 | Auxin Solar AXN6P610T250 | Auxin Solar AXN-P6T250 | Auxin Solar AXN6M610T255 | Auxin Solar AXN6P610T255 | Auxin Solar AXN-P6T255 | Auxin Solar AXN6M610T260 | Auxin Solar AXN6P610T260 | Auxin Solar AXN-P6T260 | Auxin Solar AXN6M612T265 | Auxin Solar AXN6P610T265 | Auxin Solar AXN-P6T265 | Auxin Solar AXN6M610T270 | Auxin Solar AXN6M612T270 | Auxin Solar AXN6P610T270 | Auxin Solar AXN-P6T270 | Auxin Solar AXN6M610T275 | Auxin Solar AXN6M612T275 | Auxin Solar AXN6P610T275 | Auxin Solar AXN6P612T275 | Auxin Solar AXN6P612T275G | Auxin Solar AXN-P6T275 | Auxin Solar AXN6M610T280 | Auxin Solar AXN6M612T280 | Auxin Solar AXN6P610T280 | Auxin Solar AXN6P612T280 | Auxin Solar AXN6P612T280G | Auxin Solar AXN-P6T280 | Auxin Solar AXN6M610T285 | Auxin Solar AXN6M612T285 | Auxin Solar AXN6P610T285 | Auxin Solar AXN6P612T285 | Auxin Solar AXN6P612T285G | Auxin Solar AXN-P6T285 | Auxin Solar AXN6M610T290 | Auxin Solar AXN6M612T290 | Auxin Solar AXN6P610T290 | Auxin Solar AXN6P612T290 | Auxin Solar AXN6P612T290G | Auxin Solar AXN6M610T295 | Auxin Solar AXN6M612T295 | Auxin Solar AXN6P612T295 | Auxin Solar AXN6P612T295G | Auxin Solar AXN6M610T300 | Auxin Solar AXN6M612T300 | Auxin Solar AXN6P612T300 | Auxin Solar AXN6P612T300G | Auxin Solar AXN6M610T305 | Auxin Solar AXN6M612T305 | Auxin Solar AXN6P612T305 | Auxin Solar AXN6P612T305G | Auxin Solar AXN6M610T310 | Auxin Solar AXN6M612T310 | Auxin Solar AXN6P612T310 | Auxin Solar AXN6M610T315 | Auxin Solar AXN6M612T315 | Auxin Solar AXN6P612T315 | Auxin Solar AXN6M610T320 | Auxin Solar AXN6M612T320 | Auxin Solar AXN6P612T320 | Auxin Solar AXN6M610T325 | Auxin Solar AXN6M612T325 | Auxin Solar AXN6P612T325 | Auxin Solar AXN6M612T330 | Auxin Solar AXN6P612T330 | Auxin Solar AXN6M612T335 | Auxin Solar AXN6P612T335 | Auxin Solar AXN6M612T340 | Auxin Solar AXN6M612T345 | Auxin Solar AXN6M612T350 | Auxin Solar AXN6M612T355 | Auxin Solar AXN6M612T360 | Auxin Solar AXN6M612T365 | Auxin Solar AXN6M612T370 | Auxin Solar AXN6M612T375 | Auxin Solar AXN6M612T380 | Auxin Solar AXN6M612T385 | Avancis PowerMax 100 FB | Avancis PowerMax STRONG 115 | Avancis PowerMax 120FB | Avancis PowerMax STRONG 120 | Avancis PowerMax STRONG 125 | Avancis PowerMax STRONG 130 | AXITEC AC-190M/125-72S | AXITEC AC-195M/125-72S | AXITEC AC-200M/125-72S | AXITEC AC-225P/156-60S | AXITEC AC-230M/156-60S | AXITEC AC-230P/156-60S | AXITEC AC-235M/156-60S | AXITEC AC-235P/156-60B | AXITEC AC-235P/156-60S | AXITEC AC-240M/156-60S | AXITEC AC-240P/156-60B | AXITEC AC-240P/156-60S | AXITEC AC-245M/156-60S | AXITEC AC-245P/156-60S | AXITEC AC-250M/156-60S | AXITEC AC-250P/156-60S | AXITEC AC-255M/156-60S | AXITEC AC-255P/156-60S | AXITEC AC-260M/156-60S | AXITEC AC-260P/156-60S | AXITEC AC-265M/156-60S | AXITEC AC-265P/156-60S | AXITEC AC-270M/156-60S | AXITEC AC-270P/156-60S | AXITEC AC-270P/156-72S | AXITEC AC-275P/156-72S | AXITEC AC-280M/156-60S | AXITEC AC-280P/156-72S | AXITEC AC-285M/156-60S | AXITEC AC-285M/156-72S | AXITEC AC-285P/156-72S | AXITEC AC-290M/156-60S | AXITEC AC-290M/156-72S | AXITEC AC-290P/156-72S | AXITEC AC-295M/156-72S | AXITEC AC-295P/156-72S | AXITEC AC-300M/156-72S | AXITEC AC-300P/156-72S | AXITEC AC-305M/156-72S | AXITEC AC-305P/156-72S | AXITEC AC-310M/156-72S | AXITEC AC-310P/156-72S | AXITEC AC-315M/156-72S | AXITEC AC-315P/156-72S | AXITEC AC-320P/156-72S | AXITEC AC-325P/156-72S | AXITEC AC-330P/156-72S | AXITEC AC-335P/156-72S | AXITEC AC-340M/156-72S | AXITEC AC-340P/156-72S | AXITEC AC-345M/156-72S | AXITEC AC-345P/156-72S | AXITEC AC-350M/156-72S | AXITEC AC-355M/156-72S | AxunTek Solar Energy AR931200132 | AxunTek Solar Energy AR931200134 | AxunTek Solar Energy AR931200136 | AxunTek Solar Energy AR931200138 | AxunTek Solar Energy AA963450170 | AxunTek Solar Energy AA963450175 | AxunTek Solar Energy AA963450180 | Bangkok Solar BS-52 | BannerSolar ISB20-1BSTC-90 | BannerSolar ISB20-1BSTC-95 | BannerSolar ISB20-1BSTC-100 | BannerSolar ISB20-1BSTC-105 | Baoding Tianwei Solarfilms TWSE-aSi-80W-1 | Baoding Tianwei Solarfilms TWSF-aSi-80W-1 | Baoding Tianwei Solarfilms TWSF-W-aSi-80W-1 | Baoding Tianwei Solarfilms TWSE-aSi-85W-1 | Baoding Tianwei Solarfilms TWSF-aSi-85W-1 | Baoding Tianwei Solarfilms TWSF-W-aSi-85W-1 | Baoding Tianwei Solarfilms TWSE-aSi-90W-1 | Baoding Tianwei Solarfilms TWSF-aSi-90W-1 | Baoding Tianwei Solarfilms TWSF-W-aSi-90W-1 | Baoding Tianwei Solarfilms TWSE-aSi-95W-1 | Baoding Tianwei Solarfilms TWSF-aSi-95W-1 | Baoding Tianwei Solarfilms TWSF-W-aSi-95W-1 | Baoding Tianwei Solarfilms TWSE-aSi-100W-1 | Baoding Tianwei Solarfilms TWSF-aSi-100W-1 | Baoding Tianwei Solarfilms TWSF-W-aSi-100W-1 | Beamreach Solar BR-LW-WHT-280-ABA | Beamreach Solar BR-LW-WHT-280-ABB | Beamreach Solar BR-LW-WHT-285-ABA | Beamreach Solar BR-LW-WHT-285-ABB | Beamreach Solar BR-LW-WHT-290-ABA | Beamreach Solar BR-LW-WHT-290-ABB | Beamreach Solar BR-LW-WHT-295-ABA | Beamreach Solar BR-LW-WHT-295-ABB | Beamreach Solar BR-LW-WHT-300-ABA | Beamreach Solar BR-LW-WHT-300-ABB | Beijing Zhongkexin Electronics Equipment ZKX-180D-24 | Beijing Zhongkexin Electronics Equipment ZKX-185D-24 | Beijing Zhongkexin Electronics Equipment ZKX-190D-24 | Beijing Zhongkexin Electronics Equipment ZKX-265P-24 | Beijing Zhongkexin Electronics Equipment ZKX-270P-24 | Beijing Zhongkexin Electronics Equipment ZKX-275P-24 | Beijing Zhongkexin Electronics Equipment ZKX-280P-24 | Beijing Zhongkexin Electronics Equipment ZKX-285P-24 | BIPV BIPV050-S11 | BIPV BIPV050-T11 | BIPV BIPV050-T16 | BIPV BIPV050-T86 | BIPV BIPV052-S11 | BIPV BIPV052-S16 | BIPV BIPV052-S86 | BIPV BIPV052-T11 | BIPV BIPV052-T16 | BIPV BIPV052-T86 | BIPV BIPV054-S11 | BIPV BIPV054-S16 | BIPV BIPV054-S86 | BIPV BIPV054-T16 | BIPV BIPV054-T86 | BJ Penn BJP240M-B | BJ Penn BJP245M-B | BJ Penn BJP245M-Bv | BJ Penn BJP245S-B | BJ Penn BJP250M-B | BJ Penn BJP250M-Bv | BJ Penn BJP250S-B | BJ Penn BJP255M-B | BJ Penn BJP255M-Bv | BJ Penn BJP255S-B | BJ Penn BJP260M-Bv | BJ Penn BJP265M-Bv | BJ Penn BJP270M-A | BJ Penn BJP275M-A | BJ Penn BJP280M-A | BJ Penn BJP285M-A | BJ Penn BJP285M-Av | BJ Penn BJP290M-A | BJ Penn BJP290M-Av | BJ Penn BJP295M-A | BJ Penn BJP295M-Av | BJ Penn BJP300M-A | BJ Penn BJP300M-Av | BJ Penn BJP305M-A | BJ Penn BJP305M-Av | BJ Penn BJP310M-Av | BJ Penn BJP315M-Av | Bluesun Solar Energy Tech. Co._Ltd BSM265M-60 | Bluesun Solar Energy Tech. Co._Ltd BSM270M-60 | Bluesun Solar Energy Tech. Co._Ltd BSM275M-60 | Bluesun Solar Energy Tech. Co._Ltd BSM280M-60 | Bluesun Solar Energy Tech. Co._Ltd BSM285M-60 | Bluesun Solar Energy Tech. Co._Ltd BSM290M-60 | Bluesun Solar Energy Tech. Co._Ltd BSM295M-60 | Bluesun Solar Energy Tech. Co._Ltd BSM300M-60 | Bluesun Solar Energy Tech. Co._Ltd BSM305M-60 | Bosch Solar Energy c-Si M 60-225-16 | Bosch Solar Energy c-Si M 60 NA30117 230W | Bosch Solar Energy c-Si M 60-230-16 | Bosch Solar Energy c-Si M 60 NA30117 235W | Bosch Solar Energy c-Si M 60-235-16 | Bosch Solar Energy c-Si M 60 NA30117 240W | Bosch Solar Energy c-Si M 60-240-16 | Bosch Solar Energy c-Si M60 NA30119-240Wp | Bosch Solar Energy c-Si M 60 NA30117 245W | Bosch Solar Energy c-Si M60 NA30119-245Wp | Bosch Solar Energy c-Si M60 NA42117 245W | Bosch Solar Energy c-Si M60 NA30119-250Wp | Bosch Solar Energy c-Si M60 NA42117 250W | Bosch Solar Energy c-Si M60 NA30119-255Wp | Bosch Solar Energy c-Si M60 NA42117 255W | Bosch Solar Energy c-Si M60 NA 44117 260Wp | Bosch Solar Energy c-Si M60 NA 44117 265Wp | Bosch Solar Energy c-Si M60 NA 44117 270Wp | Bosch Solar Energy c-Si P 72 NA21126 275Wp | Bosch Solar Energy c-Si P 72 NA22126 275Wp | Bosch Solar Energy c-Si P 72 NA21126 280Wp | Bosch Solar Energy c-Si P 72 NA22126 280Wp | Bosch Solar Energy c-Si P 72 NA21126 285Wp | Bosch Solar Energy c-Si P 72 NA22126 285Wp | Bosch Solar Energy c-Si M 72 NA41126 290Wp | Bosch Solar Energy c-Si P 72 NA21126 290Wp | Bosch Solar Energy c-Si P 72 NA22126 290Wp | Bosch Solar Energy c-Si M 72 NA41126 295Wp | Bosch Solar Energy c-Si P 72 NA21126 295Wp | Bosch Solar Energy c-Si P 72 NA22126 295Wp | Bosch Solar Energy c-Si M 72 NA41126 300Wp | Bosch Solar Energy c-Si M 72 NA41126 305Wp | Bosch Solar Thin Film um-Si plus 105 | Bosch Solar Thin Film um-Si plus 110 | Bosch Solar Thin Film um-Si plus 115 | Boviet Solar Technology Co._ Ltd. BVM6610P-250 | Boviet Solar Technology Co._ Ltd. BVM6610P-255 | Boviet Solar Technology Co._ Ltd. BVM6610M-260 | Boviet Solar Technology Co._ Ltd. BVM6610P-260 | Boviet Solar Technology Co._ Ltd. BVM6610M-265 | Boviet Solar Technology Co._ Ltd. BVM6610P-265 | Boviet Solar Technology Co._ Ltd. BVM6610M-270 | Boviet Solar Technology Co._ Ltd. BVM6610P-270 | Boviet Solar Technology Co._ Ltd. BVM6610M-275 | Boviet Solar Technology Co._ Ltd. BVM6610P-275 | Boviet Solar Technology Co._ Ltd. BVM6610M-280 | Boviet Solar Technology Co._ Ltd. BVM6610P-280 | Boviet Solar Technology Co._ Ltd. BVM6610M-285 | Boviet Solar Technology Co._ Ltd. BVM6610P-285 | Boviet Solar Technology Co._ Ltd. BVM6610M-290 | Boviet Solar Technology Co._ Ltd. BVM6610P-290 | Boviet Solar Technology Co._ Ltd. BVM6610M-295 | Boviet Solar Technology Co._ Ltd. BVM6610P-295 | Boviet Solar Technology Co._ Ltd. BVM6610M-300 | Boviet Solar Technology Co._ Ltd. BVM6612P-300 | Boviet Solar Technology Co._ Ltd. BVM6610M-305 | Boviet Solar Technology Co._ Ltd. BVM6612P-305 | Boviet Solar Technology Co._ Ltd. BVM6610M-310 | Boviet Solar Technology Co._ Ltd. BVM6612M-310 | Boviet Solar Technology Co._ Ltd. BVM6612P-310 | Boviet Solar Technology Co._ Ltd. BVM6610M-315 | Boviet Solar Technology Co._ Ltd. BVM6612M-315 | Boviet Solar Technology Co._ Ltd. BVM6612P-315 | Boviet Solar Technology Co._ Ltd. BVM6612M-320 | Boviet Solar Technology Co._ Ltd. BVM6612P-320 | Boviet Solar Technology Co._ Ltd. BVM6612M-325 | Boviet Solar Technology Co._ Ltd. BVM6612P-325 | Boviet Solar Technology Co._ Ltd. BVM6612M-330 | Boviet Solar Technology Co._ Ltd. BVM6612P-330 | Boviet Solar Technology Co._ Ltd. BVM6612M-335 | Boviet Solar Technology Co._ Ltd. BVM6612P-335 | Boviet Solar Technology Co._ Ltd. BVM6612M-340 | Boviet Solar Technology Co._ Ltd. BVM6612P-340 | Boviet Solar Technology Co._ Ltd. BVM6612M-345 | Boviet Solar Technology Co._ Ltd. BVM6612P-345 | Boviet Solar Technology Co._ Ltd. BVM6612M-350 | Boviet Solar Technology Co._ Ltd. BVM6612P-350 | Boviet Solar Technology Co._ Ltd. BVM6612M-355 | Boviet Solar Technology Co._ Ltd. BVM6612P-355 | Boviet Solar Technology Co._ Ltd. BVM6612M-360 | Boviet Solar Technology Co._ Ltd. BVM6612M-365 | Boviet Solar Technology Co._ Ltd. BVM6612M-370 | Boviet Solar Technology Co._ Ltd. BVM6612M-375 | Brightwatts BWI-72-P175 | Brightwatts BWI-60-M190 | Brightwatts BI-156-200W | Brightwatts BWI-60-M200 | Brightwatts BWI-60-M220 | Brightwatts BWI-96-M220 | Brightwatts BWI-60-M225 | Brightwatts BWI-96-M225 | Brightwatts BWI-60-M230 | Brightwatts BWI-96-M230 | BYD (Huizhou) Battery BYD 120P6-18 | BYD (Huizhou) Battery BYD 125P6-18 | BYD (Huizhou) Battery BYD 130P6-18 | BYD (Huizhou) Battery BYD 135P6-18 | BYD (Huizhou) Battery BYD 140P6-18 | BYD (Huizhou) Battery BYD 200P6-30 | BYD (Huizhou) Battery BYD 205P6-30 | BYD (Huizhou) Battery BYD 210P6-30 | BYD (Huizhou) Battery BYD 215P6-30 | BYD (Huizhou) Battery BYD 220P6-30 | BYD (Huizhou) Battery BYD 220P6A-30 | BYD (Huizhou) Battery BYD 225P6-30 | BYD (Huizhou) Battery BYD 225P6A-30 | BYD (Huizhou) Battery BYD 230P6-30 | BYD (Huizhou) Battery BYD 230P6A-30 | BYD (Huizhou) Battery BYD 235P6-30 | BYD (Huizhou) Battery BYD 235P6A-30 | BYD (Huizhou) Battery BYD 235P6C-30 | BYD (Huizhou) Battery BYD 240P6-30 | BYD (Huizhou) Battery BYD 240P6-36 | BYD (Huizhou) Battery BYD 240P6A-30 | BYD (Huizhou) Battery BYD 240P6C-30 | BYD (Huizhou) Battery BYD 245P6-36 | BYD (Huizhou) Battery BYD 245P6A-30 | BYD (Huizhou) Battery BYD 245P6C-30 | BYD (Huizhou) Battery BYD 250P6-36 | BYD (Huizhou) Battery BYD 250P6A-30 | BYD (Huizhou) Battery BYD 250P6C-30 | BYD (Huizhou) Battery BYD 255P6-36 | BYD (Huizhou) Battery BYD 255P6C-30 | BYD (Huizhou) Battery BYD 260P6-36 | BYD (Huizhou) Battery BYD 260P6A-36 | BYD (Huizhou) Battery BYD 265P6-36 | BYD (Huizhou) Battery BYD 265P6A-36 | BYD (Huizhou) Battery BYD 270P6-36 | BYD (Huizhou) Battery BYD 270P6A-36 | BYD (Huizhou) Battery BYD 275P6-36 | BYD (Huizhou) Battery BYD 275P6A-36 | BYD (Huizhou) Battery BYD 280P6-36 | BYD (Huizhou) Battery BYD 280P6A-36 | BYD (Huizhou) Battery BYD 280P6C-36 | BYD (Huizhou) Battery BYD 285P6-36 | BYD (Huizhou) Battery BYD 285P6A-36 | BYD (Huizhou) Battery BYD 285P6C-36 | BYD (Huizhou) Battery BYD 290P6A-36 | BYD (Huizhou) Battery BYD 290P6C-36 | BYD (Huizhou) Battery BYD 295P6A-36 | BYD (Huizhou) Battery BYD 295P6C-36 | BYD (Huizhou) Battery BYD 300P6A-36 | BYD (Huizhou) Battery BYD 300P6C-36 | BYD (Huizhou) Battery BYD 305P6C-36 | BYD Company Limited BYD 225P6C-30 | BYD Company Limited BYD 230P6C-30 | BYD Company Limited BYD 235P6C-30 | BYD Company Limited BYD 240P6C-30 | BYD Company Limited BYD 240P6C-30-DG | BYD Company Limited BYD 245P6C-30 | BYD Company Limited BYD 245P6C-30-DG | BYD Company Limited BYD245P6K-30 | BYD Company Limited BYD 250P6C-30 | BYD Company Limited BYD 250P6C-30-DG | BYD Company Limited BYD250P6K-30 | BYD Company Limited BYD 255P6C-30 | BYD Company Limited BYD 255P6C-30-DG | BYD Company Limited BYD255P6K-30 | BYD Company Limited BYD 260P6C-30 | BYD Company Limited BYD 260P6C-30-DG | BYD Company Limited BYD 260P6C-36 | BYD Company Limited BYD260P6K-30 | BYD Company Limited BYD 265P6C-30 | BYD Company Limited BYD 265P6C-30-DG | BYD Company Limited BYD 265P6C-36 | BYD Company Limited BYD265P6K-30 | BYD Company Limited BYD 270P6C-30 | BYD Company Limited BYD 270P6C-30-DG | BYD Company Limited BYD 270P6C-36 | BYD Company Limited BYD270P6K-30 | BYD Company Limited BYD 275P6C-36 | BYD Company Limited BYD275P6K-30 | BYD Company Limited BYD 280P6C-36 | BYD Company Limited BYD280P6K-30 | BYD Company Limited BYD 285P6C-36 | BYD Company Limited BYD 290P6C-36 | BYD Company Limited BYD 290P6C-36-DG | BYD Company Limited BYD 295P6C-36 | BYD Company Limited BYD 295P6C-36-DG | BYD Company Limited BYD295P6K-36 | BYD Company Limited BYD 300P6C-36 | BYD Company Limited BYD 300P6C-36-DG | BYD Company Limited BYD300P6K-36 | BYD Company Limited BYD 305P6C-36 | BYD Company Limited BYD 305P6C-36-DG | BYD Company Limited BYD305P6K-36 | BYD Company Limited BYD 310P6C-36 | BYD Company Limited BYD 310P6C-36-DG | BYD Company Limited BYD310P6K-36 | BYD Company Limited BYD 315P6C-36 | BYD Company Limited BYD 315P6C-36-DG | BYD Company Limited BYD315P6K-36 | BYD Company Limited BYD 320P6C-36-DG | BYD Company Limited BYD320P6K-36 | BYD Company Limited BYD325P6K-36 | BYD Company Limited BYD330P6K-36 | BYD Company Limited BYD335P6K-36 | BYD Company Limited BYD340P6K-36 | CA Solar MS-150M | CA Solar MS-155M | CA Solar MS-160M | CA Solar MS-165M | CA Solar MS-170M | CA Solar MS-175M | CA Solar MS-180M | Canadian Solar Inc. CS5C-80M | Canadian Solar Inc. CS5C-90M | Canadian Solar Inc. CS5T-130M | Canadian Solar Inc. CS5T-135M | Canadian Solar Inc. CS5T-140M | Canadian Solar Inc. CS6C-140P | Canadian Solar Inc. CS5T-145M | Canadian Solar Inc. CS6C-145P | Canadian Solar Inc. CS5A-150M | Canadian Solar Inc. CS5T-150M | Canadian Solar Inc. CS6A-150P | Canadian Solar Inc. CS6A-150PE | Canadian Solar Inc. CS5A-155M | Canadian Solar Inc. CS6A-155P | Canadian Solar Inc. CS6A-155PE | Canadian Solar Inc. CS5A-160M | Canadian Solar Inc. CS5A-160MX | Canadian Solar Inc. CS6A-160P | Canadian Solar Inc. CS6A-160PE | Canadian Solar Inc. CS6P-160PE | Canadian Solar Inc. CS5A-165M | Canadian Solar Inc. CS5A-165MX | Canadian Solar Inc. CS6A-165P | Canadian Solar Inc. CS6P-165PE | Canadian Solar Inc. CS5A-170M | Canadian Solar Inc. CS5A-170MX | Canadian Solar Inc. CS6A-170P | Canadian Solar Inc. CS6P-170PE | Canadian Solar Inc. CS5A-175M | Canadian Solar Inc. CS5A-175MX | Canadian Solar Inc. CS6A-175P | Canadian Solar Inc. CS6P-175PE | Canadian Solar Inc. CS5A-180M | Canadian Solar Inc. CS5A-180MX | Canadian Solar Inc. CS6A-180P | Canadian Solar Inc. CS6P-180P | Canadian Solar Inc. CS6P-180PE | Canadian Solar Inc. CS5A-185M | Canadian Solar Inc. CS5A-185MX | Canadian Solar Inc. CS6A-185P | Canadian Solar Inc. CS6P-185P | Canadian Solar Inc. CS6P-185PE | Canadian Solar Inc. CS5A-190M | Canadian Solar Inc. CS5A-190MX | Canadian Solar Inc. CS6A-190MM | Canadian Solar Inc. CS6A-190P | Canadian Solar Inc. CS6P-190P | Canadian Solar Inc. CS6P-190PE | Canadian Solar Inc. CS5A-195M | Canadian Solar Inc. CS5A-195MX | Canadian Solar Inc. CS5P-195M | Canadian Solar Inc. CS6A-195MM | Canadian Solar Inc. CS6P-195P | Canadian Solar Inc. CS6P-195PE | Canadian Solar Inc. CS5A-200M | Canadian Solar Inc. CS5P-200M | Canadian Solar Inc. CS6A-200MM | Canadian Solar Inc. CS6P-200P | Canadian Solar Inc. CS6P-200PE | Canadian Solar Inc. CS6P-200PX | Canadian Solar Inc. CS5P-205M | Canadian Solar Inc. CS6A-205MM | Canadian Solar Inc. CS6P-205M | Canadian Solar Inc. CS6P-205P | Canadian Solar Inc. CS6P-205PE | Canadian Solar Inc. CS6P-205PX | Canadian Solar Inc. CS5P-210M | Canadian Solar Inc. CS6A-210MM | Canadian Solar Inc. CS6P-210M | Canadian Solar Inc. CS6P-210P | Canadian Solar Inc. CS6P-210PE | Canadian Solar Inc. CS6P-210PX | Canadian Solar Inc. CS5P-215M | Canadian Solar Inc. CS6P-215M | Canadian Solar Inc. CS6P-215P | Canadian Solar Inc. CS6P-215PE | Canadian Solar Inc. CS6P-215PX | Canadian Solar Inc. CS5P-220M | Canadian Solar Inc. CS5P-220P | Canadian Solar Inc. CS6P-220M | Canadian Solar Inc. CS6P-220P | Canadian Solar Inc. CS6P-220PE | Canadian Solar Inc. CS6P-220PX | Canadian Solar Inc. CS5P-225M | Canadian Solar Inc. CS5P-225P | Canadian Solar Inc. CS6P-225P | Canadian Solar Inc. CS6P-225PE | Canadian Solar Inc. CS6P-225PX | Canadian Solar Inc. CS5P-230M | Canadian Solar Inc. CS5P-230P | Canadian Solar Inc. CS6P-230M | Canadian Solar Inc. CS6P-230MX | Canadian Solar Inc. CS6P-230P | Canadian Solar Inc. CS6P-230PE | Canadian Solar Inc. CS6P-230PT | Canadian Solar Inc. CS6P-230PX | Canadian Solar Inc. CS5P-235M | Canadian Solar Inc. CS5P-235P | Canadian Solar Inc. CS6P-235M | Canadian Solar Inc. CS6P-235MX | Canadian Solar Inc. CS6P-235P | Canadian Solar Inc. CS6P-235PM | Canadian Solar Inc. CS6P-235PT | Canadian Solar Inc. CS6P-235PX | Canadian Solar Inc. CS5P-240M | Canadian Solar Inc. CS5P-240P | Canadian Solar Inc. CS6P-240M | Canadian Solar Inc. CS6P-240MX | Canadian Solar Inc. CS6P-240P | Canadian Solar Inc. CS6P-240PM | Canadian Solar Inc. CS6P-240PT | Canadian Solar Inc. CS6P-240PX | Canadian Solar Inc. CS5P-245M | Canadian Solar Inc. CS6K-245P | Canadian Solar Inc. CS6K-245P-FG | Canadian Solar Inc. CS6K-245P-PG | Canadian Solar Inc. CS6P-245M | Canadian Solar Inc. CS6P-245M-EA | Canadian Solar Inc. CS6P-245MM | Canadian Solar Inc. CS6P-245MX | Canadian Solar Inc. CS6P-245P | Canadian Solar Inc. CS6P-245P-EA | Canadian Solar Inc. CS6P-245PM | Canadian Solar Inc. CS6P-245PT | Canadian Solar Inc. CS6P-245PX | Canadian Solar Inc. CS5P-250M | Canadian Solar Inc. CS6K-250M | Canadian Solar Inc. CS6K-250P | Canadian Solar Inc. CS6K-250P-FG | Canadian Solar Inc. CS6K-250P-PG | Canadian Solar Inc. CS6K-250P-SD | Canadian Solar Inc. CS6P-250M | Canadian Solar Inc. CS6P-250M-EA | Canadian Solar Inc. CS6P-250MM | Canadian Solar Inc. CS6P-250MX | Canadian Solar Inc. CS6P-250P | Canadian Solar Inc. CS6P-250P-EA | Canadian Solar Inc. CS6P-250PM | Canadian Solar Inc. CS6P-250P-SD | Canadian Solar Inc. CS6P-250PT | Canadian Solar Inc. CS6P-250PX | Canadian Solar Inc. CS5P-255M | Canadian Solar Inc. CS6K-255M | Canadian Solar Inc. CS6K-255P | Canadian Solar Inc. CS6K-255P-FG | Canadian Solar Inc. CS6K-255P-PG | Canadian Solar Inc. CS6K-255P-SD | Canadian Solar Inc. CS6P-255M | Canadian Solar Inc. CS6P-255M-EA | Canadian Solar Inc. CS6P-255MM | Canadian Solar Inc. CS6P-255MX | Canadian Solar Inc. CS6P-255P | Canadian Solar Inc. CS6P-255P-EA | Canadian Solar Inc. CS6P-255PM | Canadian Solar Inc. CS6P-255P-SD | Canadian Solar Inc. CS6P-255PX | Canadian Solar Inc. CS6X-255M | Canadian Solar Inc. CS6X-255P | Canadian Solar Inc. CS6K-260M | Canadian Solar Inc. CS6K-260M-SD | Canadian Solar Inc. CS6K-260P | Canadian Solar Inc. CS6K-260P-FG | Canadian Solar Inc. CS6K-260P-PG | Canadian Solar Inc. CS6K-260P-SD | Canadian Solar Inc. CS6P-260M | Canadian Solar Inc. CS6P-260M-EA | Canadian Solar Inc. CS6P-260MM | Canadian Solar Inc. CS6P-260MX | Canadian Solar Inc. CS6P-260P | Canadian Solar Inc. CS6P-260P-EA | Canadian Solar Inc. CS6P-260P-SD | Canadian Solar Inc. CS6P-260PX | Canadian Solar Inc. CS6X-260M | Canadian Solar Inc. CS6X-260P | Canadian Solar Inc. CS6K-265M | Canadian Solar Inc. CS6K-265P | Canadian Solar Inc. CS6K-265P-AG | Canadian Solar Inc. CS6K-265P-PG | Canadian Solar Inc. CS6K-265P-SD | Canadian Solar Inc. CS6P-265M | Canadian Solar Inc. CS6P-265MM | Canadian Solar Inc. CS6P-265MX | Canadian Solar Inc. CS6P-265P | Canadian Solar Inc. CS6P-265P-SD | Canadian Solar Inc. CS6P-265PX | Canadian Solar Inc. CS6X-265M | Canadian Solar Inc. CS6X-265P | Canadian Solar Inc. CS3K-270P-AG | Canadian Solar Inc. CS6K-270M | Canadian Solar Inc. CS6K-270M-FG | Canadian Solar Inc. CS6K-270M-SD | Canadian Solar Inc. CS6K-270P | Canadian Solar Inc. CS6K-270P-AG | Canadian Solar Inc. CS6K-270P-FG | Canadian Solar Inc. CS6K-270P-SD | Canadian Solar Inc. CS6P-270M | Canadian Solar Inc. CS6P-270MX | Canadian Solar Inc. CS6P-270P | Canadian Solar Inc. CS6P-270P-SD | Canadian Solar Inc. CS6X-270M | Canadian Solar Inc. CS6X-270P | Canadian Solar Inc. CS3K-275MS-AG | Canadian Solar Inc. CS3K-275P-AG | Canadian Solar Inc. CS6K-275M | Canadian Solar Inc. CS6K-275M-FG | Canadian Solar Inc. CS6K-275MS | Canadian Solar Inc. CS6K-275M-SD | Canadian Solar Inc. CS6K-275P | Canadian Solar Inc. CS6K-275P-AG | Canadian Solar Inc. CS6K-275P-FG | Canadian Solar Inc. CS6K-275P-SD | Canadian Solar Inc. CS6P-275M | Canadian Solar Inc. CS6P-275MX | Canadian Solar Inc. CS6P-275P | Canadian Solar Inc. CS6P-275P-SD | Canadian Solar Inc. CS6X-275M | Canadian Solar Inc. CS6X-275P | Canadian Solar Inc. CS3K-280MS-AG | Canadian Solar Inc. CS3K-280P-AG | Canadian Solar Inc. CS6K-280M | Canadian Solar Inc. CS6K-280M-FG | Canadian Solar Inc. CS6K-280MS | Canadian Solar Inc. CS6K-280M-SD | Canadian Solar Inc. CS6K-280P | Canadian Solar Inc. CS6K-280P-AG | Canadian Solar Inc. CS6P-280M | Canadian Solar Inc. CS6P-280MX | Canadian Solar Inc. CS6X-280M | Canadian Solar Inc. CS6X-280P | Canadian Solar Inc. CS3K-285MS-AG | Canadian Solar Inc. CS3K-285P-AG | Canadian Solar Inc. CS6K-285M | Canadian Solar Inc. CS6K-285M-FG | Canadian Solar Inc. CS6K-285MS | Canadian Solar Inc. CS6K-285M-SD | Canadian Solar Inc. CS6K-285P | Canadian Solar Inc. CS6K-285P-AG | Canadian Solar Inc. CS6P-285M | Canadian Solar Inc. CS6P-285MX | Canadian Solar Inc. CS6X-285M | Canadian Solar Inc. CS6X-285P | Canadian Solar Inc. CS3K-290MS-AG | Canadian Solar Inc. CS3K-290P-AG | Canadian Solar Inc. CS6K-290M | Canadian Solar Inc. CS6K-290M-FG | Canadian Solar Inc. CS6K-290MS | Canadian Solar Inc. CS6K-290P | Canadian Solar Inc. CS6X-290M | Canadian Solar Inc. CS6X-290P | Canadian Solar Inc. CS1K-295MS | Canadian Solar Inc. CS3K-295MS-AG | Canadian Solar Inc. CS3K-295P-AG | Canadian Solar Inc. CS6K-295M | Canadian Solar Inc. CS6K-295MS | Canadian Solar Inc. CS6K-295P | Canadian Solar Inc. CS6X-295M | Canadian Solar Inc. CS6X-295P | Canadian Solar Inc. CS1K-300MS | Canadian Solar Inc. CS3K-300MS-AG | Canadian Solar Inc. CS3K-300P-AG | Canadian Solar Inc. CS6K-300M | Canadian Solar Inc. CS6K-300MS | Canadian Solar Inc. CS6K-300P | Canadian Solar Inc. CS6U-300P | Canadian Solar Inc. CS6X-300M | Canadian Solar Inc. CS6X-300P | Canadian Solar Inc. CS6X-300PN | Canadian Solar Inc. CS1K-305MS | Canadian Solar Inc. CS3K-305MS-AG | Canadian Solar Inc. CS6K-305M | Canadian Solar Inc. CS6K-305MS | Canadian Solar Inc. CS6U-305P | Canadian Solar Inc. CS6X-305M | Canadian Solar Inc. CS6X-305P | Canadian Solar Inc. CS6X-305PN | Canadian Solar Inc. CS1K-310MS | Canadian Solar Inc. CS3K-310MS-AG | Canadian Solar Inc. CS3U-310P-AG | Canadian Solar Inc. CS6U-310P | Canadian Solar Inc. CS6U-310P-AG | Canadian Solar Inc. CS6X-310M | Canadian Solar Inc. CS6X-310P | Canadian Solar Inc. CS6X-310PN | Canadian Solar Inc. CS1K-315MS | Canadian Solar Inc. CS3K-315MS-AG | Canadian Solar Inc. CS3U-315P-AG | Canadian Solar Inc. CS6U-315M | Canadian Solar Inc. CS6U-315P | Canadian Solar Inc. CS6U-315P-AG | Canadian Solar Inc. CS6X-315P | Canadian Solar Inc. CS6X-315P-FG | Canadian Solar Inc. CS6X-315PN | Canadian Solar Inc. CS1K-320MS | Canadian Solar Inc. CS3K-320MS-AG | Canadian Solar Inc. CS3U-320P | Canadian Solar Inc. CS3U-320P-AG | Canadian Solar Inc. CS6U-320M | Canadian Solar Inc. CS6U-320P | Canadian Solar Inc. CS6U-320P-AG | Canadian Solar Inc. CS6X-320M-FG | Canadian Solar Inc. CS6X-320P | Canadian Solar Inc. CS6X-320P-FG | Canadian Solar Inc. CS6X-320PN | Canadian Solar Inc. CS1K-325MS | Canadian Solar Inc. CS3U-325P | Canadian Solar Inc. CS3U-325P-AG | Canadian Solar Inc. CS6U-325M | Canadian Solar Inc. CS6U-325P | Canadian Solar Inc. CS6U-325P-AG | Canadian Solar Inc. CS6X-325M-FG | Canadian Solar Inc. CS6X-325P | Canadian Solar Inc. CS6X-325P-FG | Canadian Solar Inc. CS6X-325PN | Canadian Solar Inc. CS1K-330MS | Canadian Solar Inc. CS3U-330P | Canadian Solar Inc. CS3U-330P-AG | Canadian Solar Inc. CS6U-330M | Canadian Solar Inc. CS6U-330P | Canadian Solar Inc. CS6U-330P-AG | Canadian Solar Inc. CS6X-330M-FG | Canadian Solar Inc. CS6X-330P | Canadian Solar Inc. CS6X-330P-FG | Canadian Solar Inc. CS6X-330PN | Canadian Solar Inc. CS1K-335MS | Canadian Solar Inc. CS3U-335P | Canadian Solar Inc. CS3U-335P-AG | Canadian Solar Inc. CS6U-335M | Canadian Solar Inc. CS6U-335P | Canadian Solar Inc. CS6U-335P-AG | Canadian Solar Inc. CS6X-335M-FG | Canadian Solar Inc. CS1K-340MS | Canadian Solar Inc. CS3U-340P | Canadian Solar Inc. CS3U-340P-AG | Canadian Solar Inc. CS6U-340M | Canadian Solar Inc. CS6U-340P | Canadian Solar Inc. CS6U-340P-AG | Canadian Solar Inc. CS6X-340M-FG | Canadian Solar Inc. CS3U-345P | Canadian Solar Inc. CS3U-345P-AG | Canadian Solar Inc. CS6U-345M | Canadian Solar Inc. CS6U-345P | Canadian Solar Inc. CS6X-345M-FG | Canadian Solar Inc. CS3U-350MS-AG | Canadian Solar Inc. CS3U-350P | Canadian Solar Inc. CS3U-350P-AG | Canadian Solar Inc. CS6U-350M | Canadian Solar Inc. CS6U-350P | Canadian Solar Inc. CS6X-350M-FG | Canadian Solar Inc. CS3U-355MS-AG | Canadian Solar Inc. CS3U-355P | Canadian Solar Inc. CS6U-355P | Canadian Solar Inc. CS3U-360MS-AG | Canadian Solar Inc. CS3U-360P | Canadian Solar Inc. CS6U-360P | Canadian Solar Inc. CS3U-365MS-AG | Canadian Solar Inc. CS3U-370MS-AG | Canadian Solar Inc. CS3U-375MS-AG | Caterpillar PVT105 | Caterpillar PVT105 ARC | Caterpillar PVT107 | Caterpillar PVT107 ARC | Caterpillar PVT110 | Caterpillar PVT110 ARC | Caterpillar PVT112 | Caterpillar PVT112 ARC | Caterpillar PVT115 | Caterpillar PVT115 ARC | Caterpillar PVT117 | Caterpillar PVT117 ARC | Celestica C60Q230 | Celestica C60Q230F-CT | Celestica C60Q230M | Celestica C60Q230M-Wx | Celestica C60Q235 | Celestica C60Q235F-CT | Celestica C60Q235M | Celestica C60Q235M-Wx | Celestica C60N240 | Celestica C60N240M | Celestica C60N240M-Wx | Celestica C60Q240 | Celestica C60Q240F-CT | Celestica C60Q240M | Celestica C60Q240M-Wx | Celestica C60N245 | Celestica C60N245M | Celestica C60N245M-Wx | Celestica C60Q245 | Celestica C60Q245F-CT | Celestica C60Q245M | Celestica C60Q245M-Wx | Celestica C60N250 | Celestica C60N250M | Celestica C60N250M-Wx | Celestica C60Q250 | Celestica C60Q250F-CT | Celestica C60Q250M | Celestica C60Q250M-Wx | Celestica C60N255 | Celestica C60N255L-BX | Celestica C60N255L-TX | Celestica C60N255M | Celestica C60N255M-Wx | Celestica C60Q255F-CT | Celestica C60N260 | Celestica C60N260M | Celestica C60N260M-Wx | Celestica C60Q260M-WT | Celestica C60Q260U-MT | Celestica C60N265 | Celestica C60N265M | Celestica C60N265M-Wx | Celestica C72Q280 | Celestica C72Q280M | Celestica C72Q280M-Wx | Celestica C72Q280V | Celestica C72Q280V-Wx | Celestica C72Q285 | Celestica C72Q285M | Celestica C72Q285M-Wx | Celestica C72Q285V | Celestica C72Q285V-Wx | Celestica C72N290 | Celestica C72N290M | Celestica C72N290M-Wx | Celestica C72N290V | Celestica C72N290V-Wx | Celestica C72Q290 | Celestica C72Q290M | Celestica C72Q290M-Wx | Celestica C72Q290V | Celestica C72Q290V-Wx | Celestica C72N295 | Celestica C72N295M | Celestica C72N295M-Wx | Celestica C72N295V | Celestica C72N295V-Wx | Celestica C72Q295 | Celestica C72Q295M | Celestica C72Q295M-Wx | Celestica C72Q295V | Celestica C72Q295V-Wx | Celestica C72N300 | Celestica C72N300M | Celestica C72N300M-Wx | Celestica C72N300V | Celestica C72N300V-Wx | Celestica C72Q300 | Celestica C72Q300M | Celestica C72Q300M-Wx | Celestica C72Q300V | Celestica C72Q300V-Wx | Celestica C72N305 | Celestica C72N305M | Celestica C72N305M-Wx | Celestica C72N305V | Celestica C72N305V-Wx | Celestica C72Q305 | Celestica C72Q305M | Celestica C72Q305M-Wx | Celestica C72Q305V | Celestica C72Q305V-Wx | Celestica C72N310 | Celestica C72N310M | Celestica C72N310M-Wx | Celestica C72N310V | Celestica C72N310V-Wx | Celestica C72Q310 | Celestica C72Q310M | Celestica C72Q310M-Wx | Celestica C72Q310V | Celestica C72Q310V-Wx | Celestica C72N315 | Celestica C72N315M | Celestica C72N315M-Wx | Celestica C72N315V | Celestica C72N315V-Wx | Celestica C72N320 | Celestica C72N320M | Celestica C72N320M-Wx | Celestica C72N320V | Celestica C72N320V-Wx | Centennial Solar CS200 | Centrosolar America DP36 130 | Centrosolar America DP36 135 | Centrosolar America VS-135C1 | Centrosolar America VS-135C2 | Centrosolar America DP36 140 | Centrosolar America VS-140C1 | Centrosolar America VS-140C2 | Centrosolar America DP36 145 | Centrosolar America VS-145C1 | Centrosolar America VS-145C2 | Centrosolar America DP36 150 | Centrosolar America VS-150C1 | Centrosolar America VS-150C2 | Centrosolar America VS-155C1 | Centrosolar America VS-155C2 | Centrosolar America VS-160C1 | Centrosolar America E165 | Centrosolar America E170 | Centrosolar America DP48 175 | Centrosolar America E175 | Centrosolar America DP48 180 | Centrosolar America E180 | Centrosolar America DP48 185 | Centrosolar America E185 | Centrosolar America DP48 190 | Centrosolar America DP48 195 | Centrosolar America E195 | Centrosolar America D200 | Centrosolar America DP48 200 | Centrosolar America DP54 200 | Centrosolar America E200 | Centrosolar America DP54 205 | Centrosolar America E205 | Centrosolar America D210 | Centrosolar America DP54 210 | Centrosolar America E210 | Centrosolar America DP54 215 | Centrosolar America D220 | Centrosolar America DP54 220 | Centrosolar America DP60 220 | Centrosolar America E220 | Centrosolar America E220B | Centrosolar America DP54 225 | Centrosolar America DP60 225 | Centrosolar America E225 | Centrosolar America E225B | Centrosolar America EP6 225 BW | Centrosolar America EP6 225 SW | Centrosolar America K225 | Centrosolar America K225B | Centrosolar America D230 | Centrosolar America DM60 230 | Centrosolar America DP54 230 | Centrosolar America DP60 230 | Centrosolar America E230 | Centrosolar America E230B | Centrosolar America E230BWZ | Centrosolar America E230SWZ | Centrosolar America EP6 230 BW | Centrosolar America EP6 230 SW | Centrosolar America K230 | Centrosolar America K230B | Centrosolar America BP6235BB | Centrosolar America BP6-235BW | Centrosolar America BP6235SW | Centrosolar America DM60 235 | Centrosolar America DP60 235 | Centrosolar America E235 | Centrosolar America E235B | Centrosolar America E235BWZ | Centrosolar America E235SWZ | Centrosolar America EP6 235 BW | Centrosolar America EP6 235 SW | Centrosolar America K235 | Centrosolar America K235B | Centrosolar America TUP6 235BB | Centrosolar America BP6-240BB | Centrosolar America BP6-240BW | Centrosolar America BP6-240SW | Centrosolar America DM60 240 | Centrosolar America DP60 240 | Centrosolar America E240 | Centrosolar America E240B | Centrosolar America E240BWZ | Centrosolar America E240SWZ | Centrosolar America EP6 240 BW | Centrosolar America EP6 240 SW | Centrosolar America THP6240 | Centrosolar America TUP6 240BB | Centrosolar America TUP6 240SW | Centrosolar America BP6-245BB | Centrosolar America BP6-245BW | Centrosolar America BP6-245SW | Centrosolar America DM60 245 | Centrosolar America DP60 245 | Centrosolar America E245 | Centrosolar America E245B | Centrosolar America EP6 245 BW | Centrosolar America EP6 245 SW | Centrosolar America THP6245 | Centrosolar America TP6 245xx | Centrosolar America TP6S 245xx | Centrosolar America TUP6 245BB | Centrosolar America TUP6 245SW | Centrosolar America BP6-250BB | Centrosolar America BP6-250BW | Centrosolar America BP6-250SW | Centrosolar America CM60 250xx | Centrosolar America CP60 250xx | Centrosolar America DM60 250 | Centrosolar America DP60 250 | Centrosolar America E250 | Centrosolar America E250B | Centrosolar America EP6 250BW | Centrosolar America EP6 250SW | Centrosolar America THP6250 | Centrosolar America TP6 250xx | Centrosolar America TP6S 250xx | Centrosolar America TUP6 250BB | Centrosolar America TUP6 250SW | Centrosolar America BM60 255BB | Centrosolar America BP6-255BB | Centrosolar America BP6-255BW | Centrosolar America BP6-255SW | Centrosolar America CM60 255xx | Centrosolar America DM60 255 | Centrosolar America DP60 255 | Centrosolar America E255B | Centrosolar America EP6 255BW | Centrosolar America EP6 255SW | Centrosolar America EP60 255BW | Centrosolar America EP60 255SW | Centrosolar America THP6255 | Centrosolar America TP6 255xx | Centrosolar America TP6S 255xx | Centrosolar America TUP6 255BB | Centrosolar America TUP6 255SW | Centrosolar America BM60 260BB | Centrosolar America BP6-260BB | Centrosolar America BP6-260BW | Centrosolar America BP6-260SW | Centrosolar America CM60 260BB | Centrosolar America CM60 260BW | Centrosolar America CM60 260-C1 | Centrosolar America CP60 260BB | Centrosolar America CP60 260BW | Centrosolar America CP60 260-C1 | Centrosolar America CP60 260SW | Centrosolar America DM60 260 | Centrosolar America DP60 260 | Centrosolar America E260 | Centrosolar America E260B | Centrosolar America EM60 260BB | Centrosolar America EP6 260BW | Centrosolar America EP6 260SW | Centrosolar America EP60 260BW | Centrosolar America EP60 260SW | Centrosolar America TM6 260xx | Centrosolar America TM6S 260xx | Centrosolar America TP6 260xx | Centrosolar America TP6S 260xx | Centrosolar America TUP6 260SW | Centrosolar America BM60 265BB | Centrosolar America BP6-265BB | Centrosolar America BP6-265BW | Centrosolar America BP6-265SW | Centrosolar America CM60 265BB | Centrosolar America CM60 265BW | Centrosolar America CM60 265-C1 | Centrosolar America CP60 265-C1 | Centrosolar America DM60 265 | Centrosolar America DP60 265 | Centrosolar America E265 | Centrosolar America E265B | Centrosolar America EM60 265BB | Centrosolar America EM60 265BW | Centrosolar America EM60 265SW | Centrosolar America EP6 265BW | Centrosolar America EP6 265SW | Centrosolar America EP60 265BW | Centrosolar America EP60 265SW | Centrosolar America TM6 265xx | Centrosolar America TM6S 265xx | Centrosolar America TP6 265xx | Centrosolar America TP6S 265xx | Centrosolar America BM60 270BB | Centrosolar America BP6-270BB | Centrosolar America BP6-270BW | Centrosolar America BP6-270SW | Centrosolar America CM60 270BB | Centrosolar America CM60 270BW | Centrosolar America CP60 270SW | Centrosolar America DM60 270 | Centrosolar America DP60 270 | Centrosolar America DP72 270 | Centrosolar America E270 | Centrosolar America E270B | Centrosolar America EM60 270BB | Centrosolar America EM60 270BW | Centrosolar America EM60 270SW | Centrosolar America EP60 270BW | Centrosolar America EP60 270SW | Centrosolar America TM6 270xx | Centrosolar America TM6S 270xx | Centrosolar America BM60 275BB | Centrosolar America CM60 275BB | Centrosolar America CM60 275BW | Centrosolar America CM60 275SW | Centrosolar America DM60 275 | Centrosolar America DP72 275 | Centrosolar America E275 | Centrosolar America E275B | Centrosolar America EM60 275BB | Centrosolar America EM60 275BW | Centrosolar America EM60 275SW | Centrosolar America EP60 275BW | Centrosolar America EP60 275SW | Centrosolar America EP7 275 BW | Centrosolar America EP7 275 SW | Centrosolar America SM60 275SW | Centrosolar America TM6 275xx | Centrosolar America TM6S 275xx | Centrosolar America BM60 280BB | Centrosolar America CM60 280BB | Centrosolar America CM60 280BW | Centrosolar America CM60 280SW | Centrosolar America DP72 280 | Centrosolar America E280 | Centrosolar America E280B | Centrosolar America EM60 280BB | Centrosolar America EM60 280BW | Centrosolar America EM60 280SW | Centrosolar America EP60 280BW | Centrosolar America EP60 280SW | Centrosolar America EP7 280 BW | Centrosolar America EP7 280 SW | Centrosolar America SM60 280SW | Centrosolar America TM6 280xx | Centrosolar America TM6S 280xx | Centrosolar America BM60 285BB | Centrosolar America BP7-285SW | Centrosolar America CM60 285BB | Centrosolar America CM60 285BW | Centrosolar America DM72 285 | Centrosolar America DP72 285 | Centrosolar America E285 | Centrosolar America E285B | Centrosolar America EM60 285BB | Centrosolar America EM60 285BW | Centrosolar America EM60 285SW | Centrosolar America EP7 285 BW | Centrosolar America EP7 285 SW | Centrosolar America THP7285 | Centrosolar America TM6 285xx | Centrosolar America TM6S 285xx | Centrosolar America BM60 290BB | Centrosolar America BP7-290SW | Centrosolar America CM60 290BB | Centrosolar America CM60 290BW | Centrosolar America DM72 290 | Centrosolar America DP72 290 | Centrosolar America E290 | Centrosolar America E290B | Centrosolar America EM60 290BW | Centrosolar America EM60 290SW | Centrosolar America EP7 290 BW | Centrosolar America EP7 290 SW | Centrosolar America THP7290 | Centrosolar America TP7 290xx | Centrosolar America TP7S 290xx | Centrosolar America BP7-295SW | Centrosolar America CM60 295BB | Centrosolar America CM60 295BW | Centrosolar America DM72 295 | Centrosolar America DP72 295 | Centrosolar America E295 | Centrosolar America E295B | Centrosolar America EP7 295 BW | Centrosolar America EP7 295 SW | Centrosolar America TP7 295xx | Centrosolar America TP7S 295xx | Centrosolar America BP7-300SW | Centrosolar America CM60 300BB | Centrosolar America CM60 300BW | Centrosolar America CM72 300xx | Centrosolar America CP72 300-C1 | Centrosolar America CP72 300SW | Centrosolar America DM72 300 | Centrosolar America DP72 300 | Centrosolar America E300 | Centrosolar America E300B | Centrosolar America THP7300 | Centrosolar America TP7 300xx | Centrosolar America TP7S 300xx | Centrosolar America TUP7 300SW | Centrosolar America BP7-305BW | Centrosolar America BP7-305SW | Centrosolar America CM72 305xx | Centrosolar America CP72 305-C1 | Centrosolar America CP72 305SW | Centrosolar America DM72 305 | Centrosolar America DP72 305 | Centrosolar America E305 | Centrosolar America E305B | Centrosolar America EP72 305BW | Centrosolar America EP72 305SW | Centrosolar America THP7305 | Centrosolar America TP7 305xx | Centrosolar America TP7S 305xx | Centrosolar America TUP7 305SW | Centrosolar America BP7-310BW | Centrosolar America BP7-310SW | Centrosolar America CM72 310-C1 | Centrosolar America CP72 310-C1 | Centrosolar America CP72 310SW | Centrosolar America DM72 310 | Centrosolar America DP72 310 | Centrosolar America EP72 310BW | Centrosolar America EP72 310SW | Centrosolar America THP7310 | Centrosolar America TP7 310xx | Centrosolar America TP7S 310xx | Centrosolar America TUP7 310SW | Centrosolar America BP7-315BW | Centrosolar America BP7-315SW | Centrosolar America CM72 315-C1 | Centrosolar America CP72 315-C1 | Centrosolar America CP72 315SW | Centrosolar America DM72 315 | Centrosolar America DP72 315 | Centrosolar America EP72 315BW | Centrosolar America EP72 315SW | Centrosolar America SP72 315SW | Centrosolar America THM7315 | Centrosolar America TM7 315BW | Centrosolar America TM7 315SW | Centrosolar America TM7S 315BW | Centrosolar America TM7S 315SW | Centrosolar America TP7 315xx | Centrosolar America TP7S 315xx | Centrosolar America TUP7 315SW | Centrosolar America BP7-320BW | Centrosolar America BP7-320SW | Centrosolar America CM72 320-C1 | Centrosolar America CM72 320SW | Centrosolar America CP72 320-C1 | Centrosolar America CP72 320SW | Centrosolar America DM72 320 | Centrosolar America DP72 320 | Centrosolar America EM72 320BW | Centrosolar America EM72 320SW | Centrosolar America EP72 320BW | Centrosolar America EP72 320SW | Centrosolar America SP72 320SW | Centrosolar America THM7320 | Centrosolar America TM7 320BW | Centrosolar America TM7 320SW | Centrosolar America TM7S 320BW | Centrosolar America TM7S 320SW | Centrosolar America TP7 320xx | Centrosolar America TP7S 320xx | Centrosolar America CM72 325SW | Centrosolar America CP72 325SW | Centrosolar America DM72 325 | Centrosolar America DP72 325 | Centrosolar America EM72 325BW | Centrosolar America EM72 325SW | Centrosolar America EP72 325BW | Centrosolar America EP72 325SW | Centrosolar America TM7 325BW | Centrosolar America TM7 325SW | Centrosolar America TM7S 325BW | Centrosolar America TM7S 325SW | Centrosolar America CM72 330SW | Centrosolar America CP72 330SW | Centrosolar America DM72 330 | Centrosolar America DP72 330 | Centrosolar America EM72 330BW | Centrosolar America EM72 330SW | Centrosolar America EP72 330BW | Centrosolar America EP72 330SW | Centrosolar America SM72 330SW | Centrosolar America TM7 330BW | Centrosolar America TM7 330SW | Centrosolar America TM7S 330BW | Centrosolar America TM7S 330SW | Centrosolar America CM72 335SW | Centrosolar America DM72 335 | Centrosolar America EM72 335BW | Centrosolar America EM72 335SW | Centrosolar America EP72 335BW | Centrosolar America EP72 335SW | Centrosolar America SM72 335SW | Centrosolar America TM7 335BW | Centrosolar America TM7 335SW | Centrosolar America TM7S 335BW | Centrosolar America TM7S 335SW | Centrosolar America EM72 340BW | Centrosolar America EM72 340SW | Centrosolar America SM72 340SW | Centrosolar America EM72 345BW | Centrosolar America EM72 345SW | Centrosolar America EM72 350BW | Centrosolar America EM72 350SW | Centrosolar Canada SP6 220SW | Centrosolar Canada SP6 225SW | Centrosolar Canada SP6 230SW | Centrosolar Canada SP6 235SW | Centrosolar Canada SP6 240SW | Centrosolar Canada SP6 245SW | Centrosolar Canada SP6 250SW | Centrosolar Canada SP6 255SW | Centrosolar Canada SP7 265SW | Centrosolar Canada SP7 270SW | Centrosolar Canada SP7 275SW | Centrosolar Canada SP7 280SW | Centrosolar Canada SP7 285SW | CentroSolar Sonnenstromfabrik CP6230BW | CentroSolar Sonnenstromfabrik CP6230SW | CentroSolar Sonnenstromfabrik CP6235BW | CentroSolar Sonnenstromfabrik CP6235SW | CentroSolar Sonnenstromfabrik CP6240BW | CentroSolar Sonnenstromfabrik CP6240SW | CertainTeed Apollo | CertainTeed APOLLO TILE-B | CertainTeed APOLLO TILE-G | CertainTeed Apollo II-54 | CertainTeed Apollo Tile II-54 | CertainTeed Apollo II-55 | CertainTeed Apollo Tile II-55 | CertainTeed Apollo II-56 | CertainTeed Apollo Tile II-56 | CertainTeed Apollo II-57 | CertainTeed Apollo Tile II-57 | CertainTeed Apollo II-58 | CertainTeed Apollo Tile II-58 | CertainTeed Apollo II-59 | CertainTeed Apollo Tile II-59 | CertainTeed Apollo II-60 | CertainTeed Apollo Tile II-60 | CertainTeed Apollo II-61 | CertainTeed Apollo Tile II-61 | CertainTeed Apollo II-62 | CertainTeed Apollo Tile II-62 | CertainTeed Apollo II-63 | CertainTeed Apollo Tile II-63 | CertainTeed CT260P00-01 | CertainTeed CT260P10-01 | CertainTeed CT265M11-01 | CertainTeed CT270M11-01 | CertainTeed CT280M10-02 | CertainTeed CT280M11-02 | Certainteed CT285M10-01 | CertainTeed CT285M10-02 | Certainteed CT285M11-01 | Certainteed CT290M10-01 | CertainTeed CT290M10-02 | Certainteed CT290M11-01 | CertainTeed CT290M11-02 | Certainteed CT295M10-01 | CertainTeed CT295M10-02 | Certainteed CT295M11-01 | CertainTeed CT295M11-02 | Certainteed CT300M10-01 | CertainTeed CT300M10-02 | CertainTeed CT300M10-03 | Certainteed CT300M11-01 | CertainTeed CT300M11-02 | CertainTeed CT300M11-03 | CertainTeed CT305M10-02 | CertainTeed CT305M11-02 | CertainTeed CT320P00-01 | CertainTeed CT325P00-01 | CertainTeed CT340Mz0-03 | CertainTeed CT350M00-01 | CertainTeed CT350M10-01 | CertainTeed CT355M00-01 | CertainTeed CT355M10-01 | CertainTeed CT355M10-02 | CertainTeed CT355M10-03 | CertainTeed CT355M11-02 | CertainTeed CT355M11-03 | CertainTeed CT360M00-01 | CertainTeed CT360M10-01 | CertainTeed CT360M10-02 | CertainTeed CT360M10-03 | CertainTeed CT360M11-02 | CertainTeed CT360M11-03 | CertainTeed CT365M10-02 | CertainTeed CT365M11-02 | Changzhou Almaden SEBP60S-220 | Changzhou Almaden SEBP60S-225 | Changzhou Almaden SEAP60-230 | Changzhou Almaden SEBP60S-230 | Changzhou Almaden SEAP60-235 | Changzhou Almaden SEBP60S-235 | Changzhou Almaden SEAP60-240 | Changzhou Almaden SEBP60S-240 | Changzhou Almaden SEAP60-245 | Changzhou Almaden SEBP60S-245 | Changzhou Almaden SEAP60-250 | Changzhou Almaden SEBP60S-250 | Changzhou Almaden SEAP60-255 | Changzhou Almaden SEAP60-260 | Changzhou Almaden SEAP72-280 | Changzhou Almaden SEAP72-285 | Changzhou Almaden SEAP72-290 | Changzhou Almaden SEAP72-295 | Changzhou Almaden SEAP72-300 | Changzhou Almaden SEAP72-305 | Changzhou Eging Photovoltaic Technology EGM-150 | Changzhou Eging Photovoltaic Technology EGM-155 | Changzhou Eging Photovoltaic Technology EGM-160 | Changzhou Eging Photovoltaic Technology EGM-165 | Changzhou Eging Photovoltaic Technology EG-170P48-C | Changzhou Eging Photovoltaic Technology EGM-170 | Changzhou Eging Photovoltaic Technology EG-175P48-C | Changzhou Eging Photovoltaic Technology EGM-175 | Changzhou Eging Photovoltaic Technology EG-180M48-C | Changzhou Eging Photovoltaic Technology EG-180P48-C | Changzhou Eging Photovoltaic Technology EGM-180 | Changzhou Eging Photovoltaic Technology EG-185M48-C | Changzhou Eging Photovoltaic Technology EGM-185 | Changzhou Eging Photovoltaic Technology EG-190M48-C | Changzhou Eging Photovoltaic Technology EG-190P54-C | Changzhou Eging Photovoltaic Technology EGM-190 | Changzhou Eging Photovoltaic Technology EG-195P54-C | Changzhou Eging Photovoltaic Technology EG-200P54-C | Changzhou Eging Photovoltaic Technology EG-205M54-C | Changzhou Eging Photovoltaic Technology EG-205P54-C | Changzhou Eging Photovoltaic Technology EG-210M54-C | Changzhou Eging Photovoltaic Technology EG-210P54-C | Changzhou Eging Photovoltaic Technology EG-210P60-C | Changzhou Eging Photovoltaic Technology EG-215M54-C | Changzhou Eging Photovoltaic Technology EG-215P60-C | Changzhou Eging Photovoltaic Technology EG-220P60-C | Changzhou Eging Photovoltaic Technology EG-225M60-C | Changzhou Eging Photovoltaic Technology EG-225P60-C | Changzhou Eging Photovoltaic Technology EG-230M60-C | Changzhou Eging Photovoltaic Technology EG-230P60-C | Changzhou Eging Photovoltaic Technology EG-235M60-C | Changzhou Eging Photovoltaic Technology EG-240M72-C | Changzhou Eging Photovoltaic Technology EG-245M72-C | Changzhou Eging Photovoltaic Technology EG-255P72-C | Changzhou Eging Photovoltaic Technology EG-260P72-C | Changzhou Eging Photovoltaic Technology EG-265M72-C | Changzhou Eging Photovoltaic Technology EG-265P72-C | Changzhou Eging Photovoltaic Technology EG-270M72-C | Changzhou Eging Photovoltaic Technology EG-270P72-C | Changzhou Eging Photovoltaic Technology EG-275M72-C | Changzhou Eging Photovoltaic Technology EG-275P72-C | Changzhou Eging Photovoltaic Technology EG-280M72-C | Changzhou Eging Photovoltaic Technology EG-280P72-C | Changzhou Eging Photovoltaic Technology EG-285M72-C | Changzhou Nesl Solartech DJ-165D | Changzhou Nesl Solartech DJ-170D | Changzhou Nesl Solartech DJ-175D | Changzhou Nesl Solartech DJ-180D | Changzhou Nesl Solartech DJ-185D | Changzhou Nesl Solartech DJ-190D | Changzhou Nesl Solartech DJ-195D | Changzhou Nesl Solartech DJ-200D | Changzhou Nesl Solartech DJ-200P | Changzhou Nesl Solartech DJ-210P | Changzhou Nesl Solartech DJ-220P | Changzhou Nesl Solartech DJ-230P | Changzhou Nesl Solartech DJ-230P-ST15 | Changzhou Nesl Solartech DJ-235P | Changzhou Nesl Solartech DJ-235P-ST15 | Changzhou Nesl Solartech DJ-240DA/C | Changzhou Nesl Solartech DJ-240DA/C-ST15 | Changzhou Nesl Solartech DJ-240PA | Changzhou Nesl Solartech DJ-245DA/C | Changzhou Nesl Solartech DJ-245DA/C-ST15 | Changzhou Nesl Solartech DJ-250DA/C | Changzhou Nesl Solartech DJ-250DA/C-ST15 | Changzhou Nesl Solartech DJ-250P | Changzhou Nesl Solartech DJ-255D/C | Changzhou Nesl Solartech DJ-255D/C-ST15 | Changzhou Nesl Solartech DJ-260P | Changzhou Nesl Solartech DJ-270P | Changzhou Nesl Solartech DJ-280P | Changzhou Nesl Solartech DJ-285P | Changzhou Nesl Solartech DJ-290D/C | Changzhou Nesl Solartech DJ-290P | Changzhou Nesl Solartech DJ-295D/C | Changzhou Nesl Solartech DJ-295P | Changzhou Nesl Solartech DJ-300D/C | Changzhou Nesl Solartech DJ-300P | Changzhou Nesl Solartech DJ-305D/C | Changzhou Nesl Solartech DJ-310D/C | Chi Mei Energy CSSU-100A | Chi Mei Energy CSSU-100B | China Sunergy (Nanjing) CSUN170-72M | China Sunergy (Nanjing) CSUN175-72M | China Sunergy (Nanjing) SST175-72M | China Sunergy (Nanjing) CSUN180-72M | China Sunergy (Nanjing) SST180-72M | China Sunergy (Nanjing) CSUN185-72M | China Sunergy (Nanjing) SST185-72M | China Sunergy (Nanjing) CSUN190-72M | China Sunergy (Nanjing) SST190-72M | China Sunergy (Nanjing) CSUN215-54M-BB | China Sunergy (Nanjing) SST215-54M | China Sunergy (Nanjing) SST215-54M-BB | China Sunergy (Nanjing) CSUN220-54M-BB | China Sunergy (Nanjing) SST220-54M | China Sunergy (Nanjing) SST220-54M-BB | China Sunergy (Nanjing) SST220-60M | China Sunergy (Nanjing) SST220-60P | China Sunergy (Nanjing) CSUN225-54M-BB | China Sunergy (Nanjing) SST225-54M | China Sunergy (Nanjing) SST225-54M-BB | China Sunergy (Nanjing) SST225-60M | China Sunergy (Nanjing) SST225-60P | China Sunergy (Nanjing) SST230-60M | China Sunergy (Nanjing) SST230-60P | China Sunergy (Nanjing) CSUN235-60M-BB | China Sunergy (Nanjing) CSUN235-60P-BW | China Sunergy (Nanjing) SST235-60M | China Sunergy (Nanjing) SST235-60M-BB | China Sunergy (Nanjing) SST235-60P | China Sunergy (Nanjing) SST235-60P-BW | China Sunergy (Nanjing) CSUN240-54M | China Sunergy (Nanjing) CSUN240-60M-BB | China Sunergy (Nanjing) CSUN240-60P-BW | China Sunergy (Nanjing) SST240-54M | China Sunergy (Nanjing) SST240-60M | China Sunergy (Nanjing) SST240-60M-BB | China Sunergy (Nanjing) SST240-60P | China Sunergy (Nanjing) SST240-60P-BW | China Sunergy (Nanjing) CSUN245-60M | China Sunergy (Nanjing) CSUN245-60M-BB | China Sunergy (Nanjing) CSUN245-60M-BW | China Sunergy (Nanjing) CSUN245-60P | China Sunergy (Nanjing) CSUN245-60P-BW | China Sunergy (Nanjing) SST245-60M | China Sunergy (Nanjing) SST245-60M-BB | China Sunergy (Nanjing) SST245-60M-BW | China Sunergy (Nanjing) SST245-60P | China Sunergy (Nanjing) SST245-60P-BW | China Sunergy (Nanjing) CSUN250-60M | China Sunergy (Nanjing) CSUN250-60M-BW | China Sunergy (Nanjing) CSUN250-60P | China Sunergy (Nanjing) CSUN250-60P-BW | China Sunergy (Nanjing) SST250-60M | China Sunergy (Nanjing) SST250-60M-BW | China Sunergy (Nanjing) SST250-60P | China Sunergy (Nanjing) SST250-60P-BW | China Sunergy (Nanjing) CSUN255-60M | China Sunergy (Nanjing) CSUN255-60M-BW | China Sunergy (Nanjing) CSUN255-60P | China Sunergy (Nanjing) CSUN255-60P-BW | China Sunergy (Nanjing) SST255-60M | China Sunergy (Nanjing) SST255-60M-BW | China Sunergy (Nanjing) SST255-60P | China Sunergy (Nanjing) SST255-60P-BW | China Sunergy (Nanjing) CSUN260-60M | China Sunergy (Nanjing) CSUN260-60M-BW | China Sunergy (Nanjing) CSUN260-60P | China Sunergy (Nanjing) SST260-60M | China Sunergy (Nanjing) SST260-60M-BW | China Sunergy (Nanjing) SST260-60P | China Sunergy (Nanjing) CSUN265-60M | China Sunergy (Nanjing) CSUN265-60M-BW | China Sunergy (Nanjing) CSUN265-60P | China Sunergy (Nanjing) SST265-60M | China Sunergy (Nanjing) SST265-60M-BW | China Sunergy (Nanjing) SST265-72M | China Sunergy (Nanjing) CSUN270-60M | China Sunergy (Nanjing) CSUN270-60P | China Sunergy (Nanjing) SST270-60M | China Sunergy (Nanjing) SST270-72M | China Sunergy (Nanjing) CSUN275-60M | China Sunergy (Nanjing) SST275-60M | China Sunergy (Nanjing) SST275-72M | China Sunergy (Nanjing) SST275-72P | China Sunergy (Nanjing) CSUN280-60M | China Sunergy (Nanjing) CSUN280-72M-BB | China Sunergy (Nanjing) CSUN280-72P | China Sunergy (Nanjing) SST280-60M | China Sunergy (Nanjing) SST280-72M | China Sunergy (Nanjing) SST280-72M-BB | China Sunergy (Nanjing) SST280-72P | China Sunergy (Nanjing) CSUN285-60M | China Sunergy (Nanjing) CSUN285-72M-BB | China Sunergy (Nanjing) SST285-72M | China Sunergy (Nanjing) SST285-72M-BB | China Sunergy (Nanjing) SST285-72P | China Sunergy (Nanjing) CSUN290-60M | China Sunergy (Nanjing) CSUN290-72M-BB | China Sunergy (Nanjing) CSUN290-72P | China Sunergy (Nanjing) SST290-72M | China Sunergy (Nanjing) SST290-72M-BB | China Sunergy (Nanjing) SST290-72P | China Sunergy (Nanjing) CSUN295-72M-BB | China Sunergy (Nanjing) CSUN295-72P | China Sunergy (Nanjing) SST295-72M | China Sunergy (Nanjing) SST295-72M-BB | China Sunergy (Nanjing) CSUN300-72P | China Sunergy (Nanjing) SST300-72M | China Sunergy (Nanjing) CSUN305-72M | China Sunergy (Nanjing) CSUN305-72P | China Sunergy (Nanjing) SST305-72M | China Sunergy (Nanjing) CSUN310-72M | China Sunergy (Nanjing) CSUN310-72P | China Sunergy (Nanjing) SST310-72M | China Sunergy (Nanjing) CSUN315-72M | China Sunergy (Nanjing) CSUN315-72P | China Sunergy (Nanjing) SST315-72M | China Sunergy (Nanjing) CSUN320-72M | China Sunergy (Nanjing) CSUN320-72P | China Sunergy (Nanjing) SST320-72M | China Sunergy (Nanjing) CSUN325-72M | China Sunergy (Nanjing) SST325-72M | China Sunergy (Nanjing) CSUN330-72M | China Sunergy (Nanjing) SST330-72M | China Sunergy (Nanjing) CSUN335-72M | China Sunergy (Nanjing) CSUN340-72M | China Sunergy (Nanjing) CSUN345-72M | Chinaland Solar Energy HSE235-60P | Chinaland Solar Energy HSE235-60P-B | Chinaland Solar Energy HSE240-60M | Chinaland Solar Energy HSE240-60M-B | Chinaland Solar Energy HSE240-60P | Chinaland Solar Energy HSE240-60P-B | Chinaland Solar Energy HSE245-60M | Chinaland Solar Energy HSE245-60M-B | Chinaland Solar Energy HSE245-60P | Chinaland Solar Energy HSE245-60P-B | Chinaland Solar Energy HSE250-60M | Chinaland Solar Energy HSE250-60M-B | Chinaland Solar Energy HSE250-60P | Chinaland Solar Energy HSE250-60P-B | Chinaland Solar Energy HSE255-60M | Chinaland Solar Energy HSE255-60M-B | Chinaland Solar Energy HSE255-60P | Chinaland Solar Energy HSE255-60P-B | Chinaland Solar Energy HSE260-60M | Chinaland Solar Energy HSE260-60M-B | Chinaland Solar Energy HSE260-60P | Chinaland Solar Energy HSE260-60P-B | Chinaland Solar Energy HSE265-60M | Chinaland Solar Energy HSE265-60M-B | Chinaland Solar Energy HSE265-60P | Chinaland Solar Energy HSE265-60P-B | Chinaland Solar Energy HSE270-60M | Chinaland Solar Energy HSE270-60M-B | Chinaland Solar Energy HSE270-60P | Chinaland Solar Energy HSE270-60P-B | Chinaland Solar Energy HSE275-60M-B | Chinaland Solar Energy HSE290-72P | Chinaland Solar Energy HSE295-72M | Chinaland Solar Energy HSE295-72P | Chinaland Solar Energy HSE300-72M | Chinaland Solar Energy HSE300-72P | Chinaland Solar Energy HSE305-72M | Chinaland Solar Energy HSE305-72P | Chinaland Solar Energy HSE310-72M | Chinaland Solar Energy HSE310-72P | Chinaland Solar Energy HSE315-72M | Chinaland Solar Energy HSE315-72P | Chinaland Solar Energy HSE320-72M | Chinaland Solar Energy HSE320-72P | Chinaland Solar Energy HSE325-72M | Chinalight Haoyu Photovoltaic Technology (Beijing) CLS165P | Chinalight Haoyu Photovoltaic Technology (Beijing) CLS170P | Chinalight Haoyu Photovoltaic Technology (Beijing) CLS175P | Chinalight Haoyu Photovoltaic Technology (Beijing) CLS180P | Chinalight Haoyu Photovoltaic Technology (Beijing) CLS185P | Chinalight Haoyu Photovoltaic Technology (Beijing) CLS190P | Chinalight Haoyu Photovoltaic Technology (Beijing) CLS215P | Chinalight Haoyu Photovoltaic Technology (Beijing) CLS220P | Chinalight Haoyu Photovoltaic Technology (Beijing) CLS-225P | Chinalight Haoyu Photovoltaic Technology (Beijing) CLS-230P | Chinalight Haoyu Photovoltaic Technology (Beijing) CLS-235P | Chinalight Haoyu Photovoltaic Technology (Beijing) CLS-240P | Chinalight Haoyu Photovoltaic Technology (Beijing) CLS-245P | Chinalight Haoyu Photovoltaic Technology (Beijing) CLS-250P | Chint Solar (Zhejiang) Co._ Ltd CHSM5001T-105 | Chint Solar (Zhejiang) Co._ Ltd CHSM5001T-110 | Chint Solar (Zhejiang) Co._ Ltd CHSM5001T-115 | Chint Solar (Zhejiang) Co._ Ltd CHSM5031T-125 | Chint Solar (Zhejiang) Co._ Ltd CHSM5031T-130 | Chint Solar (Zhejiang) Co._ Ltd CHSM5031T-135 | Chint Solar (Zhejiang) Co._ Ltd CHSM5612M-175 | Chint Solar (Zhejiang) Co._ Ltd CHSM5612M-180 | Chint Solar (Zhejiang) Co._ Ltd CHSM5612M(BL)-185 | Chint Solar (Zhejiang) Co._ Ltd CHSM5612M-185 | Chint Solar (Zhejiang) Co._ Ltd CHSM5612M(BL)-190 | Chint Solar (Zhejiang) Co._ Ltd CHSM5612M-190 | Chint Solar (Zhejiang) Co._ Ltd CHSM5612M(BL)-195 | Chint Solar (Zhejiang) Co._ Ltd CHSM5612M-195 | Chint Solar (Zhejiang) Co._ Ltd CHSM5612M(BL)-200 | Chint Solar (Zhejiang) Co._ Ltd CHSM5612M-200 | Chint Solar (Zhejiang) Co._ Ltd CHSM5612M-205 | Chint Solar (Zhejiang) Co._ Ltd CHSM5612M-210 | Chint Solar (Zhejiang) Co._ Ltd CHSM6609M-215 | Chint Solar (Zhejiang) Co._ Ltd CHSM6610P-215 | Chint Solar (Zhejiang) Co._ Ltd CHSM6609M-220 | Chint Solar (Zhejiang) Co._ Ltd CHSM6610M-220 | Chint Solar (Zhejiang) Co._ Ltd CHSM6610P-220 | Chint Solar (Zhejiang) Co._ Ltd CHSM6609M-225 | Chint Solar (Zhejiang) Co._ Ltd CHSM6610M-225 | Chint Solar (Zhejiang) Co._ Ltd CHSM6610P-225 | Chint Solar (Zhejiang) Co._ Ltd CHSM6609M-230 | Chint Solar (Zhejiang) Co._ Ltd CHSM6610M-230 | Chint Solar (Zhejiang) Co._ Ltd CHSM6610P-230 | Chint Solar (Zhejiang) Co._ Ltd CHSM6609M-235 | Chint Solar (Zhejiang) Co._ Ltd CHSM6610M-235 | Chint Solar (Zhejiang) Co._ Ltd CHSM6610P-235 | Chint Solar (Zhejiang) Co._ Ltd CHSM6609M-240 | Chint Solar (Zhejiang) Co._ Ltd CHSM6610M(BL)-240 | Chint Solar (Zhejiang) Co._ Ltd CHSM6610M-240 | Chint Solar (Zhejiang) Co._ Ltd CHSM6610P-240 | Chint Solar (Zhejiang) Co._ Ltd CHSM6610M(BL)-245 | Chint Solar (Zhejiang) Co._ Ltd CHSM6610M-245 | Chint Solar (Zhejiang) Co._ Ltd CHSM6610P-245 | Chint Solar (Zhejiang) Co._ Ltd CHSM6610M(BL)-250 | Chint Solar (Zhejiang) Co._ Ltd CHSM6610M-250 | Chint Solar (Zhejiang) Co._ Ltd CHSM6610P/HV-250 | Chint Solar (Zhejiang) Co._ Ltd CHSM6610P-250 | Chint Solar (Zhejiang) Co._ Ltd CHSM6610PR-250 | Chint Solar (Zhejiang) Co._ Ltd CHSM6610M(BL)-255 | Chint Solar (Zhejiang) Co._ Ltd CHSM6610M-255 | Chint Solar (Zhejiang) Co._ Ltd CHSM6610P/HV-255 | Chint Solar (Zhejiang) Co._ Ltd CHSM6610P-255 | Chint Solar (Zhejiang) Co._ Ltd CHSM6610PR-255 | Chint Solar (Zhejiang) Co._ Ltd CHSM6610M(BL)-260 | Chint Solar (Zhejiang) Co._ Ltd CHSM6610M-260 | Chint Solar (Zhejiang) Co._ Ltd CHSM6610P/HV-260 | Chint Solar (Zhejiang) Co._ Ltd CHSM6610P-260 | Chint Solar (Zhejiang) Co._ Ltd CHSM6610PR-260 | Chint Solar (Zhejiang) Co._ Ltd CHSM6612P-260 | Chint Solar (Zhejiang) Co._ Ltd CHSM6610M-265 | Chint Solar (Zhejiang) Co._ Ltd CHSM6610P/HV-265 | Chint Solar (Zhejiang) Co._ Ltd CHSM6610P-265 | Chint Solar (Zhejiang) Co._ Ltd CHSM6611P-265 | Chint Solar (Zhejiang) Co._ Ltd CHSM6612P-265 | Chint Solar (Zhejiang) Co._ Ltd CHSM6610M-270 | Chint Solar (Zhejiang) Co._ Ltd CHSM6610P/HV-270 | Chint Solar (Zhejiang) Co._ Ltd CHSM6610P-270 | Chint Solar (Zhejiang) Co._ Ltd CHSM6611P-270 | Chint Solar (Zhejiang) Co._ Ltd CHSM6612P-270 | Chint Solar (Zhejiang) Co._ Ltd CHSM6610M/HV-275 | Chint Solar (Zhejiang) Co._ Ltd CHSM6610M-275 | Chint Solar (Zhejiang) Co._ Ltd CHSM6610P/HV-275 | Chint Solar (Zhejiang) Co._ Ltd CHSM6610P-275 | Chint Solar (Zhejiang) Co._ Ltd CHSM6611P-275 | Chint Solar (Zhejiang) Co._ Ltd CHSM6612P-275 | Chint Solar (Zhejiang) Co._ Ltd CHSM6612PM-275 | Chint Solar (Zhejiang) Co._ Ltd CHSM6610M(BL)-280 | Chint Solar (Zhejiang) Co._ Ltd CHSM6610M/HV-280 | Chint Solar (Zhejiang) Co._ Ltd CHSM6610M-280 | Chint Solar (Zhejiang) Co._ Ltd CHSM6610P/HV-280 | Chint Solar (Zhejiang) Co._ Ltd CHSM6610P-280 | Chint Solar (Zhejiang) Co._ Ltd CHSM6611P-280 | Chint Solar (Zhejiang) Co._ Ltd CHSM6612P-280 | Chint Solar (Zhejiang) Co._ Ltd CHSM6612PM-280 | Chint Solar (Zhejiang) Co._ Ltd CHSM6610M(BL)-285 | Chint Solar (Zhejiang) Co._ Ltd CHSM6610M/HV-285 | Chint Solar (Zhejiang) Co._ Ltd CHSM6610M-285 | Chint Solar (Zhejiang) Co._ Ltd CHSM6610P/HV-285 | Chint Solar (Zhejiang) Co._ Ltd CHSM6610P-285 | Chint Solar (Zhejiang) Co._ Ltd CHSM6611P-285 | Chint Solar (Zhejiang) Co._ Ltd CHSM6612P-285 | Chint Solar (Zhejiang) Co._ Ltd CHSM6612PM-285 | Chint Solar (Zhejiang) Co._ Ltd CHSM6610M(BL)-290 | Chint Solar (Zhejiang) Co._ Ltd CHSM6610M/HV-290 | Chint Solar (Zhejiang) Co._ Ltd CHSM6610M-290 | Chint Solar (Zhejiang) Co._ Ltd CHSM6610P/HV-290 | Chint Solar (Zhejiang) Co._ Ltd CHSM6610P-290 | Chint Solar (Zhejiang) Co._ Ltd CHSM6612P-290 | Chint Solar (Zhejiang) Co._ Ltd CHSM6612PM-290 | Chint Solar (Zhejiang) Co._ Ltd CHSM6610M(BL)-295 | Chint Solar (Zhejiang) Co._ Ltd CHSM6610M/HV-295 | Chint Solar (Zhejiang) Co._ Ltd CHSM6610M-295 | Chint Solar (Zhejiang) Co._ Ltd CHSM6610P/HV-295 | Chint Solar (Zhejiang) Co._ Ltd CHSM6610P-295 | Chint Solar (Zhejiang) Co._ Ltd CHSM6612M-295 | Chint Solar (Zhejiang) Co._ Ltd CHSM6612P-295 | Chint Solar (Zhejiang) Co._ Ltd CHSM6612PM-295 | Chint Solar (Zhejiang) Co._ Ltd CHSM6612PR-295 | Chint Solar (Zhejiang) Co._ Ltd CHSM6610M/HV-300 | Chint Solar (Zhejiang) Co._ Ltd CHSM6612M-300 | Chint Solar (Zhejiang) Co._ Ltd CHSM6612P-300 | Chint Solar (Zhejiang) Co._ Ltd CHSM6612PR-300 | Chint Solar (Zhejiang) Co._ Ltd CHSM6610M/HV-305 | Chint Solar (Zhejiang) Co._ Ltd CHSM6612M-305 | Chint Solar (Zhejiang) Co._ Ltd CHSM6612P-305 | Chint Solar (Zhejiang) Co._ Ltd CHSM6612PR-305 | Chint Solar (Zhejiang) Co._ Ltd CHSM6612M-310 | Chint Solar (Zhejiang) Co._ Ltd CHSM6612P/HV-310 | Chint Solar (Zhejiang) Co._ Ltd CHSM6612P-310 | Chint Solar (Zhejiang) Co._ Ltd CHSM6612M-315 | Chint Solar (Zhejiang) Co._ Ltd CHSM6612P/HV-315 | Chint Solar (Zhejiang) Co._ Ltd CHSM6612P-315 | Chint Solar (Zhejiang) Co._ Ltd CHSM6612M-320 | Chint Solar (Zhejiang) Co._ Ltd CHSM6612P/HV-320 | Chint Solar (Zhejiang) Co._ Ltd CHSM6612P-320 | Chint Solar (Zhejiang) Co._ Ltd CHSM6612M-325 | Chint Solar (Zhejiang) Co._ Ltd CHSM6612P/HV-325 | Chint Solar (Zhejiang) Co._ Ltd CHSM6612P-325 | Chint Solar (Zhejiang) Co._ Ltd CHSM6612M(BL)-330 | Chint Solar (Zhejiang) Co._ Ltd CHSM6612M/HV-330 | Chint Solar (Zhejiang) Co._ Ltd CHSM6612M-330 | Chint Solar (Zhejiang) Co._ Ltd CHSM6612P/HV-330 | Chint Solar (Zhejiang) Co._ Ltd CHSM6612P-330 | Chint Solar (Zhejiang) Co._ Ltd CHSM6612M(BL)-335 | Chint Solar (Zhejiang) Co._ Ltd CHSM6612M/HV-335 | Chint Solar (Zhejiang) Co._ Ltd CHSM6612M-335 | Chint Solar (Zhejiang) Co._ Ltd CHSM6612P/HV-335 | Chint Solar (Zhejiang) Co._ Ltd CHSM6612P-335 | Chint Solar (Zhejiang) Co._ Ltd CHSM6612M(BL)-340 | Chint Solar (Zhejiang) Co._ Ltd CHSM6612M/HV-340 | Chint Solar (Zhejiang) Co._ Ltd CHSM6612M-340 | Chint Solar (Zhejiang) Co._ Ltd CHSM6612P/HV-340 | Chint Solar (Zhejiang) Co._ Ltd CHSM6612P-340 | Chint Solar (Zhejiang) Co._ Ltd CHSM6612M(BL)-345 | Chint Solar (Zhejiang) Co._ Ltd CHSM6612M/HV-345 | Chint Solar (Zhejiang) Co._ Ltd CHSM6612M-345 | Chint Solar (Zhejiang) Co._ Ltd CHSM6612P/HV-345 | Chint Solar (Zhejiang) Co._ Ltd CHSM6612P-345 | Chint Solar (Zhejiang) Co._ Ltd CHSM6612M(BL)-350 | Chint Solar (Zhejiang) Co._ Ltd CHSM6612M/HV-350 | Chint Solar (Zhejiang) Co._ Ltd CHSM6612M-350 | Chint Solar (Zhejiang) Co._ Ltd CHSM6612P/HV-350 | Chint Solar (Zhejiang) Co._ Ltd CHSM6612M(BL)-355 | Chint Solar (Zhejiang) Co._ Ltd CHSM6612M/HV-355 | Chint Solar (Zhejiang) Co._ Ltd CHSM6612M-355 | Chint Solar (Zhejiang) Co._ Ltd CHSM6612P/HV-355 | Chint Solar (Zhejiang) Co._ Ltd CHSM6612M(BL)-360 | Chint Solar (Zhejiang) Co._ Ltd CHSM6612M/HV-360 | Chint Solar (Zhejiang) Co._ Ltd CHSM6612M-360 | Clean Source & Energy CSE115M-1 | Clean Source & Energy CSE120M-1 | Clean Source & Energy CSE125M-1 | Clean Source & Energy CSE150M-2 | Clean Source & Energy CSE155M-2 | Clean Source & Energy CSE160M-1 | Clean Source & Energy CSE160M-2 | Clean Source & Energy CSE165M-1 | Clean Source & Energy CSE165M-2 | Clean Source & Energy CSE170M-1 | Clean Source & Energy CSE170M-2 | Clean Source & Energy CSE175M-1 | Clean Source & Energy CSE175M-2 | Clean Source & Energy CSE180M-1 | Clean Source & Energy CSE180M-2 | Clean Source & Energy CSE180M-3 | Clean Source & Energy CSE185M-1 | Clean Source & Energy CSE185M-2 | Clean Source & Energy CSE190P-3 | Clean Source & Energy CSE195P-3 | Clean Source & Energy CSE200M-2 | Clean Source & Energy CSE200P-1 | Clean Source & Energy CSE200P-2 | Clean Source & Energy CSE200P-3 | Clean Source & Energy CSE205M-2 | Clean Source & Energy CSE205P-1 | Clean Source & Energy CSE205P-2 | Clean Source & Energy CSE205P-3 | Clean Source & Energy CSE210M-2 | Clean Source & Energy CSE210P-1 | Clean Source & Energy CSE210P-2 | Clean Source & Energy CSE215M-2 | Clean Source & Energy CSE215P-1 | Clean Source & Energy CSE215P-2 | Clean Source & Energy CSE220M-2 | Clean Source & Energy CSE220P-1 | Clean Source & Energy CSE220P-2 | Clean Source & Energy CSE220P-3 | Clean Source & Energy CSE220P-AS | Clean Source & Energy CSE225M-2 | Clean Source & Energy CSE225M-AS | Clean Source & Energy CSE225P-2 | Clean Source & Energy CSE225P-3 | Clean Source & Energy CSE230M-2 | Clean Source & Energy CSE230P-2 | Clean Source & Energy CSE230P-3 | Clean Source & Energy CSE230P-AS | Clean Source & Energy CSE235M-2 | Clean Source & Energy CSE235M-AS | Clean Source & Energy CSE240M-2 | Clean Source & Energy CSE250P-3 | Clean Source & Energy CSE255P-3 | Clean Source & Energy CSE270P-3 | Clean Source & Energy CSE275P-3 | Clean Source & Energy CSE280P-3 | CNBM International CNBM175SAb | CNBM International CNBM175SAb(Black) | CNBM International CNBM180SAb | CNBM International CNBM180SAb(Black) | CNBM International CNBM185SAb | CNBM International CNBM185SAb(Black) | CNBM International CNBM220PCe | CNBM International CNBM220PCe(Black) | CNBM International CNBM225PCe | CNBM International CNBM225PCe(Black) | CNBM International CNBM230PCe | CNBM International CNBM230PCe(Black) | CNBM International CNBM235PCe | CNBM International CNBM235PCe(Black) | CNBM International CNBM240PCe | CNBM International CNBM240PCe(Black) | CNPV Dongying Solar Power CNPV-170M | CNPV Dongying Solar Power CNPV-175M | CNPV Dongying Solar Power CNPV-180M | CNPV Dongying Solar Power CNPV-185M | CNPV Dongying Solar Power CNPV-190M | CNPV Dongying Solar Power CNPV-195M | CNPV Dongying Solar Power CNPV-200M | CNPV Dongying Solar Power CNPV-200P-54 | CNPV Dongying Solar Power CNPV-205M | CNPV Dongying Solar Power CNPV-205P-54 | CNPV Dongying Solar Power CNPV-210M-54 | CNPV Dongying Solar Power CNPV-210P-54 | CNPV Dongying Solar Power CNPV-215M-54 | CNPV Dongying Solar Power CNPV-215P-54 | CNPV Dongying Solar Power CNPV-220M-54 | CNPV Dongying Solar Power CNPV-220P-54 | CNPV Dongying Solar Power CNPV-225M-54 | CNPV Dongying Solar Power CNPV-225P | CNPV Dongying Solar Power CNPV-225P-54 | CNPV Dongying Solar Power CNPV-230M-54 | CNPV Dongying Solar Power CNPV-230P | CNPV Dongying Solar Power CNPV-230P-54 | CNPV Dongying Solar Power CNPV-235P | CNPV Dongying Solar Power CNPV-235P-54 | CNPV Dongying Solar Power CNPV-240M | CNPV Dongying Solar Power CNPV-240P | CNPV Dongying Solar Power CNPV-245M | CNPV Dongying Solar Power CNPV-245P | CNPV Dongying Solar Power CNPV-250M | CNPV Dongying Solar Power CNPV-250P | CNPV Dongying Solar Power CNPV-255M | CNPV Dongying Solar Power CNPV-255P | CNPV Dongying Solar Power CNPV-260M | CNPV Dongying Solar Power CNPV-260P | CNPV Dongying Solar Power CNPV-270P | CNPV Dongying Solar Power CNPV-275M | CNPV Dongying Solar Power CNPV-275P | CNPV Dongying Solar Power CNPV-280M | CNPV Dongying Solar Power CNPV-280P | CNPV Dongying Solar Power CNPV-285M | CNPV Dongying Solar Power CNPV-285P | CNPV Dongying Solar Power CNPV-290M | CNPV Dongying Solar Power CNPV-290P | CNPV Dongying Solar Power CNPV-295M | CNPV Dongying Solar Power CNPV-295P | CNPV Dongying Solar Power CNPV-300M | CNPV Dongying Solar Power CNPV-300P | CNPV Dongying Solar Power CNPV-305M | CNPV Dongying Solar Power CNPV-305P | CNPV Dongying Solar Power CNPV-310M | CNPV Dongying Solar Power CNPV-310P | CNPV Dongying Solar Power CNPV-315P | Cogenra Solar TC-M300 | Cogenra Solar TC-M310 | Conergy Conergy Black 170M | Conergy Conergy P 170M | Conergy Conergy Black 175M | Conergy Conergy P 175M | Conergy Conergy PH 175M | Conergy Conergy Black 180M | Conergy Conergy P 180M | Conergy Conergy Black 185M | Conergy Conergy P 185M | Conergy Conergy P 190P | Conergy Conergy P 195P | Conergy Conergy P 200P | Conergy Conergy P 205P | Conergy Conergy Black 210PA | Conergy Conergy P 210P | Conergy Conergy P 210PA | Conergy Conergy Black 215PA | Conergy Conergy P 215PA | Conergy Conergy Black 220PA | Conergy Conergy P 220PA | Conergy Conergy PH 220P | Conergy Conergy PM 220P | Conergy Conergy Black 225PA | Conergy Conergy P 225PA | Conergy Conergy PH 225P | Conergy Conergy PM 225P | Conergy Conergy Black 230PA | Conergy Conergy P 230PA | Conergy Conergy PH 230M | Conergy Conergy PH 230P | Conergy Conergy PM 230P | Conergy Conergy Black 235PA | Conergy Conergy P 235PA | Conergy Conergy PH 235M | Conergy Conergy PH 235P | Conergy Conergy PM 235P | Conergy Conergy PH 240M | Conergy Conergy PH 240M BL | Conergy Conergy PH 240P | Conergy Conergy PM 240P | Conergy Conergy PE 245P | Conergy Conergy PH 245M | Conergy Conergy PH 245M BL | Conergy Conergy PH 245P | Conergy Conergy PM 245P | Conergy Conergy PE 250P | Conergy Conergy PH 250M | Conergy Conergy PH 250M BL | Conergy Conergy PH 250P | Conergy Conergy PM 250P | Conergy Conergy PE 255P | Conergy Conergy PH 255M | Conergy Conergy PH 255M BL | Conergy Conergy PH 255P | Conergy Conergy PM 255P | Conergy Conergy PE 260P | Conergy Conergy PH 260M | Conergy Conergy PH 260P | Conergy Conergy PM 260P | Conergy Conergy PH 285P | Conergy Conergy PH 290P | Conergy Conergy PE 295P | Conergy Conergy PH 295P | Conergy Conergy PE 300P | Conergy Conergy PH 300P | Conergy Conergy PE 305P | Conergy Conergy PH 305P | Conergy Conergy PE 310P | Conergy Conergy PH 310P | Conergy Holding CONERGY ON 220-60 | Conergy Holding CONERGY ON 225-60 | Conergy Holding CONERGY ON 230-60 | Conergy Holding CONERGY ON 235-60 | Conergy Holding CONERGY ON 240-60 | Conergy Holding CONERGY ON 245-60 | Conergy Holding CONERGY ON 250-60 | Conergy Holding CONERGY ON 255-60 | Conergy Holding CONERGY ON 265P-72 | Conergy Holding CONERGY ON 270P-72 | Conergy Holding CONERGY ON 275P-72 | Conergy Holding CONERGY ON 280P-72 | Conergy Holding CONERGY ON 285P-72 | Conergy Solarmodule PowerPlus 215P | Conergy Solarmodule PowerPlus 220P | Conergy Solarmodule PowerPlus 225P | Cosmos Energy SL195-18 | Cosmos Energy SL200-18 | Cosmos Energy SL205-18 | Cosmos Energy SL220-20 | Cosmos Energy SL225-20 | Cosmos Energy SL230-20 | CSG PVTech CSG160M2-24 | CSG PVTech CSG165M2-24 | CSG PVTech CSG170M2-24 | CSG PVTech CSG175M2-24 | CSG PVTech CSG175S1-36 | CSG PVTech CSG180M2-24 | CSG PVTech CSG180S1-36 | CSG PVTech CSG185S1 | CSG PVTech CSG190M2-27 | CSG PVTech CSG190S1 | CSG PVTech CSG195M2-27 | CSG PVTech CSG195S1 | CSG PVTech CSG200M2-27 | CSG PVTech CSG205M2-27 | CSG PVTech CSG220M2-30 | CSG PVTech CSG225M2-30 | CSG PVTech CSG230M2-30 | CSG PVTech CSG235M2 | CSG PVTech CSG235S2 | CSG PVTech CSG240M2 | CSG PVTech CSG240S2 | CSG PVTech CSG245M2 | CSG PVTech CSG245S2 | CSG PVTech CSG250M2-35 | CSG PVTech CSG250S2 | CSG PVTech CSG255M2-35 | CSG PVTech CSG255S2 | CSG PVTech CSG260M2-35 | CSG PVTech CSG260S2 | CSG PVTech CSG265M2-35 | CSG PVTech CSG265S2 | CSG PVTech CSG270M2-36 | CSG PVTech CSG275M2-36 | CSG PVTech CSG280M2-36 | CSG PVTech CSG285M2 | CSG PVTech CSG285S2 | CSG PVTech CSG290M2 | CSG PVTech CSG290S2 | CSG PVTech CSG295M2 | CSG PVTech CSG295S2 | CSG PVTech CSG300M2 | CSG PVTech CSG300S2 | CSG PVTech CSG305S2 | CSUN Eurasia Energy Systems Industry and Trade CSUN255-60P | CSUN Eurasia Energy Systems Industry and Trade CSUN260-60P | CSUN Eurasia Energy Systems Industry and Trade CSUN265-60P | CSUN Eurasia Energy Systems Industry and Trade CSUN270-60M | CSUN Eurasia Energy Systems Industry and Trade CSUN270-60P | CSUN Eurasia Energy Systems Industry and Trade CSUN275-60M | CSUN Eurasia Energy Systems Industry and Trade CSUN275-60P | CSUN Eurasia Energy Systems Industry and Trade CSUN280-60M | CSUN Eurasia Energy Systems Industry and Trade CSUN285-60M | CSUN Eurasia Energy Systems Industry and Trade CSUN290-60M | CSUN Eurasia Energy Systems Industry and Trade CSUN295-60M | CSUN Eurasia Energy Systems Industry and Trade CSUN305-72P | CSUN Eurasia Energy Systems Industry and Trade CSUN310-72P | CSUN Eurasia Energy Systems Industry and Trade CSUN315-72P | CSUN Eurasia Energy Systems Industry and Trade CSUN320-72M | CSUN Eurasia Energy Systems Industry and Trade CSUN320-72P | CSUN Eurasia Energy Systems Industry and Trade CSUN325-72M | CSUN Eurasia Energy Systems Industry and Trade CSUN325-72P | CSUN Eurasia Energy Systems Industry and Trade CSUN330-72M | CSUN Eurasia Energy Systems Industry and Trade CSUN330-72P | CSUN Eurasia Energy Systems Industry and Trade CSUN 335-72M | CSUN Eurasia Energy Systems Industry and Trade CSUN340-72M | CSUN Eurasia Energy Systems Industry and Trade CSUN350-72M | Cuantum Solar SUNPORT 275P | Day4 Energy Day448MC 155 | Day4 Energy Day448MC 160 | Day4 Energy Day448MC 165 | Day4 Energy Day448MC 170 | Day4 Energy Day448MC 175 | Day4 Energy Day448MC 180 | Day4 Energy Day448MC 185 | Day4 Energy Day448MC 190 | Day4 Energy Day4 60MC-I 205 | Day4 Energy Day4 60MC-I 210 | Day4 Energy Day4 60MC-I 215 | Day4 Energy Day4 60MC-I 220 | Day4 Energy Day4 60MC-I 225 | Day4 Energy Day4 60MC-I 230 | Day4 Energy Day4 60MC-I 235 | Day4 Energy Day4 60MC-I 240 | Day4 Energy Day4 60MC-I 245 | Day4 Energy Day4 60MC-I 250 | DJ Solar DJS175S125M-72 | DJ Solar DJS180S125M-72 | DJ Solar DJS-T180S6ST | DJ Solar DJS185S125M-72 | DJ Solar DJS-T185S6ST | DJ Solar DJS190S125M-72 | DJ Solar DJS-T190S6ST | DJ Solar DJS195S125M-72 | DJ Solar DJS-T195S648ST | DJ Solar DJS-T200S648ST | DJ Solar DJS-T205S6ST | DJ Solar DJS210S156P-60 | DJ Solar DJS-T210P6PT | DJ Solar DJS-T210S6ST | DJ Solar DJS215S156P-60 | DJ Solar DJS-T215P6PT | DJ Solar DJS-T215S6ST | DJ Solar DJS220S156P-60 | DJ Solar DJS-T220P6PT | DJ Solar DJS-T220S6ST | DJ Solar DJS225S156P-60 | DJ Solar DJS-T225P6PT | DJ Solar DJS-T225S654ST | DJ Solar DJS230S156P-60 | DJ Solar DJS-T230P6PT | DJ Solar DJS235S156P-60 | DJ Solar DJS-T235S6ST | DJ Solar DJS-TU235PT | DJ Solar DJS240S156P-60 | DJ Solar DJS-T240P6PT | DJ Solar DJS-T240PT | DJ Solar DJS-T240S6ST | DJ Solar DJS-T250P6PT | DJ Solar DJS-T245P660PT | DJ Solar DJS-T245P6PT | DJ Solar DJS-T245S6ST | DJ Solar DJS-T250P660PT | DJ Solar DJS-T250ST | DJ Solar DJS-T255P666PT | DJ Solar DJS-T255P6PT | DJ Solar DJS-T260P666PT | DJ Solar DJS-T260P6PT | DJ Solar DJS-T260S6ST | DJ Solar DJS-T265P666PT | DJ Solar DJS-T265P6PT | DJ Solar DJS-T265S666ST | DJ Solar DJS-T270P666PT | DJ Solar DJS-T270P6PT | DJ Solar DJS-T270S666ST | DJ Solar DJS-T275P6PT | DJ Solar DJS-T275S666ST | DJ Solar DJS-T280P6PT | DJ Solar DJS-T280S6ST | DJ Solar DJS-T285P6PT | DJ Solar DJS-T285S6ST | DJ Solar DJS-T290P672PT | DJ Solar DJS-T290S6ST | DJ Solar DJS-T295P672PT | DJ Solar DJS-T295S6ST | DJ Solar DJS-T300P672PT | DJ Solar DJS-T300S6ST | DJ Solar DJS-T305S6ST | Dmsolar DM160M2-24 | Dmsolar DM-M160 | Dmsolar DM165M2-24 | Dmsolar DM170M2-24 | Dmsolar DM-M170 | Dmsolar DM175M2-24 | Dmsolar DM175S1-36 | Dmsolar DM180M2-24 | Dmsolar DM180S1-36 | Dmsolar DM-M180 | Dmsolar DM190M2-27 | Dmsolar DM195M2-27 | Dmsolar DM200M2-27 | Dmsolar DM-P200 | Dmsolar DM205M2-27 | Dmsolar DM-P210 | Dmsolar DM220M2-30 | Dmsolar DM-M220 | Dmsolar DM-P220 | Dmsolar DM225M2-30 | Dmsolar DM230M2-30 | Dmsolar DM-M230 | Dmsolar DM-P230 | Dmsolar DM-M240 | Dmsolar DM250M2-35 | Dmsolar DM255M2-35 | Dmsolar DM260M2-35 | Dmsolar DM265M2-35 | Dmsolar DM270M2-36 | Dmsolar DM275M2-36 | Dmsolar DM280M2-36 | Dongfang Electric (Yixing) MAGI MGSM-235-60 | Dongfang Electric (Yixing) MAGI MGSM-240-60 | Dongfang Electric (Yixing) MAGI MGSM-245-60 | Dongfang Electric (Yixing) MAGI MGSM-250-60 | Dongfang Electric (Yixing) MAGI MGSM-255-60 | Dongfang Electric (Yixing) MAGI MGSM-285-72 | Dongfang Electric (Yixing) MAGI MGSM-290-72 | Dongfang Electric (Yixing) MAGI MGSM-295-72 | Dongfang Electric (Yixing) MAGI MGSM-300-72 | Dongfang Electric (Yixing) MAGI MGSM-305-72 | Dongfang Electric (Yixing) MAGI MGSM-310-72 | Dongfang Electric (Yixing) MAGI MGSM-315-72 | Dow Chemical DPS-10-1000 | Dow Chemical DPS-12-1000 | Dow Chemical DPS-13-1000 | Dow Chemical PH 2.0-32 | Dow Chemical PH 2.0-34 | Dow Chemical PH 2.0-36 | Dow Chemical PH 2.0-37 | Dow Chemical PH 2.0-38 | Dow Chemical PH 2.0-39 | Dow Chemical PH 2.0-40 | Dow Chemical PH 2.0-41 | Dow Chemical PH 2.0-42 | Dow Chemical PH 2.0-43 | Du Pont Apollo DA095-A2 | Du Pont Apollo DA095-A6 | Du Pont Apollo DA100-A2 | Du Pont Apollo DA100-A6 | Du Pont Apollo DA102-A6 | Du Pont Apollo DA105-A2 | Du Pont Apollo DA105-A6 | Du Pont Apollo DA130-C2 | Du Pont Apollo DA133-C2 | Du Pont Apollo DA136-C2 | DuCal Solar Technology LLC DST265M-60 | DuCal Solar Technology LLC DST270M-60 | DuCal Solar Technology LLC DST275M-60 | DuCal Solar Technology LLC DST280M-60 | DuCal Solar Technology LLC DST285M-60 | DuCal Solar Technology LLC DST290M-60 | DuCal Solar Technology LLC DST295M-60 | DuCal Solar Technology LLC DST300M-60 | DuCal Solar Technology LLC DST305M-60 | DuraComm DCS-6P-36-130 | DuraComm DCS-6P-36-135 | DuraComm DCS-6P-36-140 | DuraComm DCS-6P-36-145 | DuraComm DCS-6P-36-150 | DuraComm DCS-6P-48-175 | DuraComm DCS-6P-48-180 | DuraComm DCS-6P-48-185 | DuraComm DCS-6P-48-190 | DuraComm DCS-6P-48-195 | DuraComm DCS-6P-48-200 | DuraComm DCS-6P-54-200 | DuraComm DCS-6P-54-205 | DuraComm DCS-6P-54-210 | DuraComm DCS-6P-54-215 | DuraComm DCS-6P-54-220 | DuraComm DCS-6P-60-220 | DuraComm DCS-6P-54-225 | DuraComm DCS-6P-60-225 | DuraComm DCS-6P-54-230 | DuraComm DCS-6P-60-230 | DuraComm DCS-6P-60-235 | DuraComm DCS-6P-60-240 | DuraComm DCS-6P-60-245 | DuraComm DCS-6P-60-250 | DuraComm DCS-6P-60-255 | DuraComm DCS-6P-72-265 | DuraComm DCS-6P-72-270 | DuraComm DCS-6P-72-275 | DuraComm DCS-6P-72-280 | DuraComm DCS-6P-72-285 | DuraComm DCS-6P-72-290 | DuraComm DCS-6P-72-295 | DuraComm DCS-6P-72-300 | DuraComm DCS-6P-72-305 | E&H EHS3-228 | E&H EHS3-230 | E&H EHS3-233 | E&H EHS3-235 | E&H EHS3-238 | E&H EHS3-240 | E&H EHS3-243 | E&H EHS3-245 | E&H EHS3-248 | E&H EHS3-250 | Eclipsall Energy NRG60-230M-BK | Eclipsall Energy NRG60-235M-BK | Eclipsall Energy NRG60-240M | Eclipsall Energy NRG60-240M-BK | Eclipsall Energy NRG60-240P | Eclipsall Energy NRG60-245M | Eclipsall Energy NRG60-245M-BK | Eclipsall Energy NRG60-245P | Eclipsall Energy NRG60-250M | Eclipsall Energy NRG60-250M-BK | Eclipsall Energy NRG60-250P | Eclipsall Energy NRG60-255M | Eclipsall Energy NRG60-255P | Eclipsall Energy NRG60-260M | Eclipsall Energy NRG72-290M | Eclipsall Energy NRG72-290P | Eclipsall Energy NRG72-295M | Eclipsall Energy NRG72-295P | Eclipsall Energy NRG72-300M | Eclipsall Energy NRG72-300P | Eclipsall Energy NRG72-305M | Eclipsall Energy NRG72-305P | Eclipsall Energy NRG72-310M | Eclipsall Energy NRG72-310P | Eclipsall Energy NRG72-315M | Eclipsall Energy NRG72-320M | ECO Future ECO-180C | ECO Future ECO-185C | ECO Future ECO-190C | ECO Future ECO-200P54 | ECO Future ECO-210C54 | ECO Future ECO-210P54 | ECO Future ECO-220C54 | ECO Future ECO-220P54 | ECO Future ECO-220P60 | ECO Future ECO-230C54 | ECO Future ECO-230C60 | ECO Future ECO-230P60 | ECO Future ECO-240C60 | ECO Future ECO-240P60 | ECO Future ECO-250C60 | ECO Future ECO-270P72 | ECO Future ECO-280C72 | ECO Future ECO-280P72 | ECO Future ECO-290C72 | ECO Future ECO-290P72 | ECO Future ECO-300C72 | Econess Energy EN125M-72-185 | Econess Energy EN125M-72-190 | Econess Energy EN125M-72-195 | Econess Energy EN125M-72-200 | Econess Energy EN156M-60-235 | Econess Energy EN156P-60-235 | Econess Energy EN156M-60-240 | Econess Energy EN156P-60-240 | Econess Energy EN125M-96-245 | Econess Energy EN156M-60-245 | Econess Energy EN156P-60-245 | Econess Energy EN125M-96-250 | Econess Energy EN156M-60-250 | Econess Energy EN156P-60-250 | Econess Energy EN125M-96-255 | Econess Energy EN125M-96-260 | Econess Energy EN125M-96-265 | Econess Energy EN156M-72-280 | Econess Energy EN156P-72-280 | Econess Energy EN156M-72-285 | Econess Energy EN156P-72-285 | Econess Energy EN156M-72-290 | Econess Energy EN156P-72-290 | Econess Energy EN156M-72-295 | Econess Energy EN156P-72-295 | Econess Energy EN156M-72-300 | Econess Energy EN156P-72-300 | Ecosol PV Tech ECS195P-54 | Ecosol PV Tech ECS200P-54 | Ecosol PV Tech ECS205P-54 | Ecosol PV Tech ECS220P-60 | Ecosol PV Tech ECS225P-60 | Ecosol PV Tech ECS230P-60 | EcoSolargy TWES-(155)72M | EcoSolargy ECO160A125M-72 | EcoSolargy TWES-(160)72M | EcoSolargy ECO165A125M-72 | EcoSolargy SDM-170/(165)-72M | EcoSolargy TWES-(165)72M | EcoSolargy ECO170A125M-72 | EcoSolargy SDM-170/(170)-72M | EcoSolargy TWES-(170)72M | EcoSolargy ECO175A125M-72 | EcoSolargy SDM-170/(175)-72M | EcoSolargy TWES-(175)72M | EcoSolargy ECO180A125M-72 | EcoSolargy SDM-170/(180)-72M | EcoSolargy TWES-(180)72M | EcoSolargy ECO185A125M-72 | EcoSolargy ECO185S156P-54 | EcoSolargy SDM-170/(185)-72M | EcoSolargy ECO190A125M-72 | EcoSolargy ECO190S156P-54 | EcoSolargy ECO195A125M-72 | EcoSolargy ECO195S156P-54 | EcoSolargy ECO200A125M-72 | EcoSolargy ECO200S156P-54 | EcoSolargy ECO200S156P-60 | EcoSolargy TWES-(200)60P | EcoSolargy ECO205S156P-54 | EcoSolargy ECO205S156P-60 | EcoSolargy TWES-(205)60P | EcoSolargy ECO210S156P-54 | EcoSolargy ECO210S156P-60 | EcoSolargy TWES-(210)60P | EcoSolargy ECO215S156P-54 | EcoSolargy ECO215S156P-60 | EcoSolargy TWES-(215)60P | EcoSolargy ECO220S156P-54 | EcoSolargy ECO220S156P-60 | EcoSolargy TWES-(220)60P | EcoSolargy ECO225S156P-54 | EcoSolargy ECO225S156P-60 | EcoSolargy TWES-(225)60P | EcoSolargy ECO230A156M-60 | EcoSolargy ECO230A156P-60 | EcoSolargy ECO230A156PB-60 | EcoSolargy ECO230S156M-60 | EcoSolargy ECO230S156P-54 | EcoSolargy ECO230S156P-60 | EcoSolargy TWES-(230)60P | EcoSolargy ECO235A156M-60 | EcoSolargy ECO235A156P-60 | EcoSolargy ECO235A156PB-60 | EcoSolargy ECO235S156P-60 | EcoSolargy TWES-(235)60P | EcoSolargy ECO240A156M-60 | EcoSolargy ECO240A156P-60 | EcoSolargy ECO240A156PB-60 | EcoSolargy ECO240S156M-60 | EcoSolargy ECO240S156P-60 | EcoSolargy ECO240S156P-72 | EcoSolargy ECO240T156P-60 | EcoSolargy ECO245A156M-60 | EcoSolargy ECO245A156P-60 | EcoSolargy ECO245S156P-60 | EcoSolargy ECO245S156P-72 | EcoSolargy ECO245T156P-60 | EcoSolargy ECO250A156M-60 | EcoSolargy ECO250A156P-60 | EcoSolargy ECO250H156P-60 | EcoSolargy ECO250S156M-60 | EcoSolargy ECO250S156P-60 | EcoSolargy ECO250S156P-72 | EcoSolargy ECO250T156M4-60 | EcoSolargy ECO250T156M-60 | EcoSolargy ECO250T156P-60 | EcoSolargy ECO255H156P-60 | EcoSolargy ECO255S156P-60 | EcoSolargy ECO255S156P-72 | EcoSolargy ECO255T156M4-60 | EcoSolargy ECO255T156M-60 | EcoSolargy ECO255T156P-60 | EcoSolargy ECO260H156P-60 | EcoSolargy ECO260S156P-60 | EcoSolargy ECO260S156P-72 | EcoSolargy ECO260T156M4-60 | EcoSolargy ECO260T156M-60 | EcoSolargy ECO260T156P-60 | EcoSolargy ECO265H156P-60 | EcoSolargy ECO265S156P-72 | EcoSolargy ECO265T156M4-60 | EcoSolargy ECO265T156M-60 | EcoSolargy ECO265T156P-60 | EcoSolargy ECO270H156P-60 | EcoSolargy ECO270S156P-72 | EcoSolargy ECO270T156M4-60 | EcoSolargy ECO270T156M-60 | EcoSolargy ECO270T156P-60 | EcoSolargy ECO275A156M-72 | EcoSolargy ECO275A156P-72 | EcoSolargy ECO275H156P-60 | EcoSolargy ECO275S156P-72 | EcoSolargy ECO275T156M4-60 | EcoSolargy ECO275T156M-60 | EcoSolargy ECO275T156P-60 | EcoSolargy ECO280A156M-72 | EcoSolargy ECO280A156P-72 | EcoSolargy ECO280S156P-72 | EcoSolargy ECO280T156M4-60 | EcoSolargy ECO280T156M-60 | EcoSolargy ECO280T156P-60 | EcoSolargy ECO285A156M-72 | EcoSolargy ECO285A156P-72 | EcoSolargy ECO285H156P-72 | EcoSolargy ECO285S156P-72 | EcoSolargy ECO285T156M4-60 | EcoSolargy ECO285T156M-60 | EcoSolargy ECO285T156P-60 | EcoSolargy ECO285T156P-72 | EcoSolargy ECO290A156M-72 | EcoSolargy ECO290A156P-72 | EcoSolargy ECO290H156P-72 | EcoSolargy ECO290S156P-72 | EcoSolargy ECO290T156M4-60 | EcoSolargy ECO290T156M-60 | EcoSolargy ECO290T156P-72 | EcoSolargy ECO295A156M-72 | EcoSolargy ECO295A156P-72 | EcoSolargy ECO295H156P-72 | EcoSolargy ECO295S156P-72 | EcoSolargy ECO295T156M4-60 | EcoSolargy ECO295T156M-60 | EcoSolargy ECO295T156P-72 | EcoSolargy ECO300A156M-72 | EcoSolargy ECO300H156P-72 | EcoSolargy ECO300S156P-72 | EcoSolargy ECO300T156M4-72 | EcoSolargy ECO300T156M-72 | EcoSolargy ECO300T156P-72 | EcoSolargy ECO305H156P-72 | EcoSolargy ECO305T156M4-72 | EcoSolargy ECO305T156M-72 | EcoSolargy ECO305T156P-72 | EcoSolargy ECO310H156P-72 | EcoSolargy ECO310T156M4-72 | EcoSolargy ECO310T156M-72 | EcoSolargy ECO310T156P-72 | EcoSolargy ECO315H156P-72 | EcoSolargy ECO315T156M4-72 | EcoSolargy ECO315T156M-72 | EcoSolargy ECO315T156P-72 | EcoSolargy ECO320H156P-72 | EcoSolargy ECO320T156M4-72 | EcoSolargy ECO320T156M-72 | EcoSolargy ECO320T156P-72 | EcoSolargy ECO325H156P-72 | EcoSolargy ECO325T156M4-72 | EcoSolargy ECO325T156M-72 | EcoSolargy ECO325T156P-72 | EcoSolargy ECO330T156M4-72 | EcoSolargy ECO330T156M-72 | EcoSolargy ECO330T156P-72 | EcoSolargy ECO335T156M4-72 | EcoSolargy ECO335T156M-72 | EcoSolargy ECO335T156P-72 | EcoSolargy ECO340T156M4-72 | EcoSolargy ECO340T156M-72 | EcoSolargy ECO340T156P-72 | EcoSolargy ECO345T156M4-72 | EcoSolargy ECO345T156M-72 | EcoSolargy ECO350T156M4-72 | EcoSolargy ECO350T156M-72 | EcoSolargy ECO355T156M4-72 | EcoSolargy ECO355T156M-72 | ENN Solar Energy EST-110 | ENN Solar Energy EST-115A | ENN Solar Energy EST-115 | ENN Solar Energy EST-120 | ENN Solar Energy EST-220V | ENN Solar Energy EST-228HA | ENN Solar Energy EST-228VA | ENN Solar Energy EST-230V | ENN Solar Energy EST-240V | ENN Solar Energy EST-460 | ENN Solar Energy EST-460A | Enp Sonne Solar Technikk ENP-M165MO | Enp Sonne Solar Technikk ENP-M170MO | Enp Sonne Solar Technikk ENP-M175MO | Enp Sonne Solar Technikk ENP-M180MO | Eoplly New Energy Technology EP125M/72-180W | Eoplly New Energy Technology EP125M/72-185W | Eoplly New Energy Technology EP125M/72-190W | Eoplly New Energy Technology EP125M/72-195W | Eoplly New Energy Technology EP125M/72-200W | Eoplly New Energy Technology EP125M/72-205W | Eoplly New Energy Technology EP125M/72-210W | Eoplly New Energy Technology EP156P/60-225S AC | Eoplly New Energy Technology EP156P/60-225W | Eoplly New Energy Technology EP156M/60-230S AC | Eoplly New Energy Technology EP156M/60-230W | Eoplly New Energy Technology EP156MB/60-230S AC | Eoplly New Energy Technology EP156MB/60-230W | Eoplly New Energy Technology EP156P/60-230S AC | Eoplly New Energy Technology EP156P/60-230W | Eoplly New Energy Technology EP156M/60-235S AC | Eoplly New Energy Technology EP156M/60-235W | Eoplly New Energy Technology EP156MB/60-235S AC | Eoplly New Energy Technology EP156MB/60-235W | Eoplly New Energy Technology EP156P/60-235S AC | Eoplly New Energy Technology EP156P/60-235W | Eoplly New Energy Technology EP156M/60-240S AC | Eoplly New Energy Technology EP156M/60-240W | Eoplly New Energy Technology EP156MB/60-240 AC | Eoplly New Energy Technology EP156MB/60-240S AC | Eoplly New Energy Technology EP156MB/60-240W | Eoplly New Energy Technology EP156P/60-240 AC | Eoplly New Energy Technology EP156P/60-240S AC | Eoplly New Energy Technology EP156P/60-240W | Eoplly New Energy Technology EP156M/60-245S AC | Eoplly New Energy Technology EP156M/60-245W | Eoplly New Energy Technology EP156MB/60-245 AC | Eoplly New Energy Technology EP156MB/60-245S AC | Eoplly New Energy Technology EP156MB/60-245W | Eoplly New Energy Technology EP156P/60-245 AC | Eoplly New Energy Technology EP156P/60-245S AC | Eoplly New Energy Technology EP156P/60-245W | Eoplly New Energy Technology EP156M/60-250 AC | Eoplly New Energy Technology EP156M/60-250S AC | Eoplly New Energy Technology EP156M/60-250W | Eoplly New Energy Technology EP156MB/60-250S AC | Eoplly New Energy Technology EP156MB/60-250W | Eoplly New Energy Technology EP156P/60-250S AC | Eoplly New Energy Technology EP156P/60-250W | Eoplly New Energy Technology EP156M/60-255 AC | Eoplly New Energy Technology EP156M/60-255S AC | Eoplly New Energy Technology EP156M/60-255W | Eoplly New Energy Technology EP156P/60-255S AC | Eoplly New Energy Technology EP156P/60-255W | Eoplly New Energy Technology EP156M/60-260 AC | Eoplly New Energy Technology EP156M/60-260S AC | Eoplly New Energy Technology EP156M/60-260W | Eoplly New Energy Technology EP156P/60-260S AC | Eoplly New Energy Technology EP156P/60-260W | Eoplly New Energy Technology EP156P/72-260W | Eoplly New Energy Technology EP156P/72-265W | Eoplly New Energy Technology EP156P/72-270W | Eoplly New Energy Technology EP156P/72-275W | Eoplly New Energy Technology EP156P/72-280W | Eoplly New Energy Technology EP156P/72-285W | Eoplly New Energy Technology EP156M/72-290W | Eoplly New Energy Technology EP156P/72-290W | Eoplly New Energy Technology EP156M/72-295W | Eoplly New Energy Technology EP156P/72-295W | Eoplly New Energy Technology EP156M/72-300W | Eoplly New Energy Technology EP156P/72-300W | Eoplly New Energy Technology EP156M/72-305W | Eoplly New Energy Technology EP156P/72-305W | Eoplly New Energy Technology EP156M/72-310W | Eoplly New Energy Technology EP156P/72-310W | Eoplly New Energy Technology EP156M/72-315W | Eoplly New Energy Technology EP156P/72-315W | Eoplly New Energy Technology EP156M/72-320W | Eoplly New Energy Technology EP156P/72-320W | EPV SOLAR EPV-40 | EPV SOLAR EPV-42 | ERA Solar ESPSA-170 | ERA Solar ESPSA-175 | ERA Solar ESPSA-180 | ERA Solar ESPSA-185 | ERA Solar ESPSA-190 | ERA Solar ESPSA-195 | ERA Solar ESPMC-205 | ERA Solar ESPMC-210 | ERA Solar ESPMC-215 | ERA Solar ESPMC-220 | ERA Solar ESPMC-225 | ERA Solar ESPMC-230 | ERA Solar ESPMC-235 | ERA Solar ESPMC-240 | ERA Solar ESPMC-245 | E-solar ESP6-72-295/SI | E-solar ESP6-72-300/SI | E-solar ESP6-72-305/SI | E-solar ESP6-72-310/SI | E-solar ESP6-72-315/SI | E-solar ESP6-72-320/SI | E-solar ESP6-72-325/SI | ET Solar Industry ET-M572165WW | ET Solar Industry ET-M572165WWZ | ET Solar Industry ET-M572170WW | ET Solar Industry ET-M572170WWZ | ET Solar Industry ET-M572175BB | ET Solar Industry ET-M572175BBZ | ET Solar Industry ET-M572175WW | ET Solar Industry ET-M572175WWZ | ET Solar Industry ET-M572180BB | ET Solar Industry ET-M572180BBZ | ET Solar Industry ET-M572180WW | ET Solar Industry ET-M572180WWZ | ET Solar Industry ET-M572185BB | ET Solar Industry ET-M572185BBZ | ET Solar Industry ET-M572185WW | ET Solar Industry ET-M572185WWZ | ET Solar Industry ET-M572190BBZ | ET Solar Industry ET-M572190WB | ET Solar Industry ET-M572190WW | ET Solar Industry ET-M572190WWZ | ET Solar Industry ET-P654190WB | ET Solar Industry ET-P654190WW | ET Solar Industry ET-P654195WB | ET Solar Industry ET-P654195WW | ET Solar Industry ET-P654200WB | ET Solar Industry ET-P654200WW | ET Solar Industry ET-P654205WB | ET Solar Industry ET-P654205WW | ET Solar Industry ET-P654210WB | ET Solar Industry ET-P654210WW | ET Solar Industry ET-P660220WB | ET Solar Industry ET-P660220WBZ | ET Solar Industry ET-P660220WW | ET Solar Industry ET-P660220WWZ | ET Solar Industry ET-A-P660225 | ET Solar Industry ET-A-P660225B | ET Solar Industry ET-P660225WB | ET Solar Industry ET-P660225WBZ | ET Solar Industry ET-P660225WW | ET Solar Industry ET-P660225WWZ | ET Solar Industry ET-A-P660230 | ET Solar Industry ET-A-P660230B | ET Solar Industry ET-P660230B | ET Solar Industry ET-P660230WB | ET Solar Industry ET-P660230WBZ | ET Solar Industry ET-P660230WW | ET Solar Industry ET-P660230WWZ | ET Solar Industry ET-A-M660235 | ET Solar Industry ET-A-M660235B | ET Solar Industry ET-A-P660235 | ET Solar Industry ET-A-P660235B | ET Solar Industry ET-P660235B | ET Solar Industry ET-P660235BB | ET Solar Industry ET-P660235BBZ | ET Solar Industry ET-P660235WB | ET Solar Industry ET-P660235WBZ | ET Solar Industry ET-P660235WW | ET Solar Industry ET-P660235WWZ | ET Solar Industry ET-A-M660240 | ET Solar Industry ET-A-M660240B | ET Solar Industry ET-A-P660240 | ET Solar Industry ET-A-P660240B | ET Solar Industry ET-M660240BB | ET Solar Industry ET-M660240WW | ET Solar Industry ET-P660240B | ET Solar Industry ET-P660240BB | ET Solar Industry ET-P660240BBZ | ET Solar Industry ET-P660240WB | ET Solar Industry ET-P660240WBZ | ET Solar Industry ET-P660240WW | ET Solar Industry ET-P660240WWZ | ET Solar Industry ET-A-M660245 | ET Solar Industry ET-A-M660245B | ET Solar Industry ET-A-P660245 | ET Solar Industry ET-A-P660245B | ET Solar Industry ET-M660245BB | ET Solar Industry ET-M660245WW | ET Solar Industry ET-P660245B | ET Solar Industry ET-P660245BAC | ET Solar Industry ET-P660245BB | ET Solar Industry ET-P660245BBAC | ET Solar Industry ET-P660245BBZ | ET Solar Industry ET-P660245BBZAC | ET Solar Industry ET-P660245WB | ET Solar Industry ET-P660245WBZ | ET Solar Industry ET-P660245WBZAC | ET Solar Industry ET-P660245WW | ET Solar Industry ET-P660245WWZ | ET Solar Industry ET-A-M660250 | ET Solar Industry ET-A-M660250B | ET Solar Industry ET-M660250BB | ET Solar Industry ET-M660250WW | ET Solar Industry ET-P660250BAC | ET Solar Industry ET-P660250BB | ET Solar Industry ET-P660250BBAC | ET Solar Industry ET-P660250BBZ | ET Solar Industry ET-P660250BBZAC | ET Solar Industry ET-P660250WB | ET Solar Industry ET-P660250WBAC | ET Solar Industry ET-P660250WBZ | ET Solar Industry ET-P660250WBZAC | ET Solar Industry ET-P660250WW | ET Solar Industry ET-P660250WWZ | ET Solar Industry ET-P672250 | ET Solar Industry ET-A-M660255 | ET Solar Industry ET-A-M660255B | ET Solar Industry ET-M660255BB | ET Solar Industry ET-M660255WW | ET Solar Industry ET-P660255BB | ET Solar Industry ET-P660255BBAC | ET Solar Industry ET-P660255BBZ | ET Solar Industry ET-P660255BBZAC | ET Solar Industry ET-P660255WB | ET Solar Industry ET-P660255WBAC | ET Solar Industry ET-P660255WBZ | ET Solar Industry ET-P660255WBZAC | ET Solar Industry ET-P660255WW | ET Solar Industry ET-P660255WWAC | ET Solar Industry ET-P660255WWZ | ET Solar Industry ET-P660255WWZAC | ET Solar Industry ET-P672255 | ET Solar Industry ET-A-M660260 | ET Solar Industry ET-A-M660260B | ET Solar Industry ET-M660260BB | ET Solar Industry ET-M660260WW | ET Solar Industry ET-P660260WB | ET Solar Industry ET-P660260WBAC | ET Solar Industry ET-P660260WBZ | ET Solar Industry ET-P660260WBZAC | ET Solar Industry ET-P660260WW | ET Solar Industry ET-P660260WWAC | ET Solar Industry ET-P660260WWZ | ET Solar Industry ET-P660260WWZAC | ET Solar Industry ET-P672260WB | ET Solar Industry ET-P672260WW | ET Solar Industry ET-A-M660265 | ET Solar Industry ET-A-M660265B | ET Solar Industry ET-M660265BB | ET Solar Industry ET-M660265WB | ET Solar Industry ET-M660265WW | ET Solar Industry ET-P660265WB | ET Solar Industry ET-P660265WW | ET Solar Industry ET-P672265WB | ET Solar Industry ET-P672265WW | ET Solar Industry ET-M660270BB | ET Solar Industry ET-M660270WB | ET Solar Industry ET-M660270WW | ET Solar Industry ET-P660270WB | ET Solar Industry ET-P660270WW | ET Solar Industry ET-P672270WB | ET Solar Industry ET-P672270WW | ET Solar Industry ET-A-P672275 | ET Solar Industry ET-A-P672275B | ET Solar Industry ET-M660275BB | ET Solar Industry ET-M660275WB | ET Solar Industry ET-M660275WW | ET Solar Industry ET-P660275WB | ET Solar Industry ET-P660275WW | ET Solar Industry ET-P672275WB | ET Solar Industry ET-P672275WW | ET Solar Industry ET-A-P672280 | ET Solar Industry ET-A-P672280B | ET Solar Industry ET-M660280BB | ET Solar Industry ET-M660280WB | ET Solar Industry ET-M660280WW | ET Solar Industry ET-P660280WB | ET Solar Industry ET-P660280WW | ET Solar Industry ET-P672280WB | ET Solar Industry ET-P672280WBG | ET Solar Industry ET-P672280WW | ET Solar Industry ET-P672280WWG | ET Solar Industry ET-A-M672285 | ET Solar Industry ET-A-M672285B | ET Solar Industry ET-A-P672285 | ET Solar Industry ET-A-P672285B | ET Solar Industry ET-M660285BB | ET Solar Industry ET-M660285WB | ET Solar Industry ET-M660285WW | ET Solar Industry ET-P672285WB | ET Solar Industry ET-P672285WBG | ET Solar Industry ET-P672285WW | ET Solar Industry ET-P672285WWG | ET Solar Industry ET-A-M672290 | ET Solar Industry ET-A-M672290B | ET Solar Industry ET-A-P672290 | ET Solar Industry ET-A-P672290B | ET Solar Industry ET-M660290WB | ET Solar Industry ET-M660290WW | ET Solar Industry ET-P672290WB | ET Solar Industry ET-P672290WBG | ET Solar Industry ET-P672290WW | ET Solar Industry ET-P672290WWG | ET Solar Industry ET-A-M672295 | ET Solar Industry ET-A-M672295B | ET Solar Industry ET-A-P672295 | ET Solar Industry ET-A-P672295B | ET Solar Industry ET-P672295WB | ET Solar Industry ET-P672295WBG | ET Solar Industry ET-P672295WW | ET Solar Industry ET-P672295WWG | ET Solar Industry ET-A-M672300 | ET Solar Industry ET-A-M672300B | ET Solar Industry ET-P672300WB | ET Solar Industry ET-P672300WBG | ET Solar Industry ET-P672300WW | ET Solar Industry ET-P672300WWG | ET Solar Industry ET-A-M672305 | ET Solar Industry ET-A-M672305B | ET Solar 